simulink model "g1_walking"  (R2025b)
settings: Solver=daessc  StartTime=0.0  StopTime=4.8  MaxStep=0.0005  RelTol=1e-6  AbsTol=1e-8
model workspace (MAT data in the model file):
  g1_base_p0 = [0; 0; 0.8]
  g1_base_rpy0 = [0; 0; 0]
  g1_command_height = 0.8
  g1_forward_command = 0.1
  g1_gravity = [0 0 -9.81]
  g1_q0 = [-0.05 0 0 -0.05 0 0 0.1 0 0 0 0 0 ... (29 elements, 29x1)]
  g1_qd0 = [0 0 0 0 0 0 0 0 0 0 0 0 ... (29 elements, 29x1)]
  g1_standing = 0
values from neighbouring files (symbols this model uses):
  g1_action_Ts = 0.002    [g1_data.sldd]
  g1_contact_threshold = 1.0    [g1_data.sldd]
  g1_cop_threshold = 5.0    [g1_data.sldd]
  g1_drive_Ts = 0.0005    [g1_data.sldd]
  g1_ground_height = 0.0    [g1_data.sldd]
  g1_limits = -0.87267 -0.2618 -1.0472 -2.5307 -0.5236 -2.7576 -0.087267 -3.0892 -1.5882 -2.618 -1.614429558 -1.972222054 -1.614429558 -0.87267 -0.2618 -1.0472 -2.5307 -2.9671 -2.7576 -0.087267 -3.0892 -2.2515 -2.618 -1.614429558 -1.972222054 -1.614429558 -0.52 -0.52 -2.618 0.5236 0.2618 2.0944 2.8798 2.9671 2.7576 2.8798 2.6704 2.2515 2.618 1.614429558 1.972222054 1.614429558 0.5236 0.2618 2.0944 2.8798 0.5236    [g1_data.sldd]
  g1_tau_max = 50.0 50.0 25.0 88.0 88.0 88.0 139.0 25.0 25.0 25.0 5.0 25.0 5.0 50.0 50.0 25.0 88.0 88.0 88.0 139.0 25.0 25.0 25.0 5.0 25.0 5.0 50.0 50.0 88.0    [g1_data.sldd]
undefined symbols (not defined in the file or in its folder): X, Y, Z
libraries: sm_lib x336, nesl_utility x122, simulink x1
(part 2 of 7)

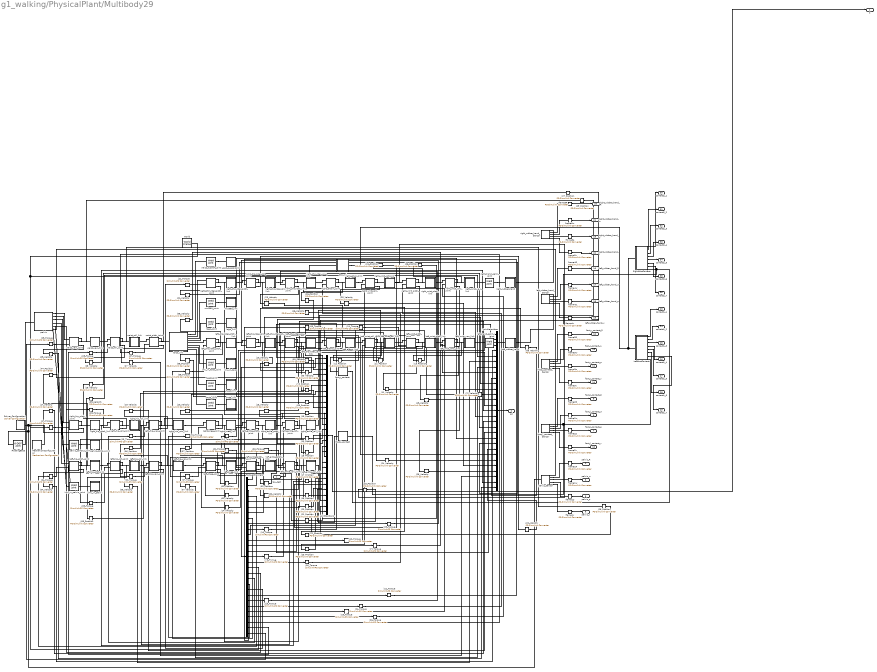
== system g1_walking/PhysicalPlant/Multibody29 ==
  tau_test : Inport  PortDimensions=29
  FloatingBase : sm_lib/Joints/6-DOF Joint  JointMode=Normal  CompositeWrenchDir=FollowerOnBase  CompositeWrenchFrame=BaseFrame  SenseConstraintForce=off  SenseConstraintTorque=off  SenseTotalForce=off  SenseTotalTorque=off  PxPositionTargetSpecify=on  PxPositionTargetPriority=High  PxPositionTargetValue=g1_base_p0(1)  PxPositionTargetValueUnits=m  PxVelocityTargetSpecify=on  PxVelocityTargetPriority=High  PxVelocityTargetValue=0  PxVelocityTargetValueUnits=m/s  PxEquilibriumPosition=0  PxEquilibriumPositionUnits=m  PxSpringStiffness=0  PxSpringStiffnessUnits=N/m  PxDampingCoefficient=0  PxDampingCoefficientUnits=N/(m/s)  PxLowerLimitSpecify=off  PxLowerLimitBound=-1  PxLowerLimitBoundUnits=m  PxLowerLimitStiffness=1e6  PxLowerLimitStiffnessUnits=N/m  PxLowerLimitDamping=1e3  PxLowerLimitDampingUnits=N/(m/s)  PxLowerLimitTransitionRegionWidth=1e-4  PxLowerLimitTransitionRegionWidthUnits=m  PxUpperLimitSpecify=off  PxUpperLimitBound=1  PxUpperLimitBoundUnits=m  PxUpperLimitStiffness=1e6  PxUpperLimitStiffnessUnits=N/m  PxUpperLimitDamping=1e3  PxUpperLimitDampingUnits=N/(m/s)  PxUpperLimitTransitionRegionWidth=1e-4  PxUpperLimitTransitionRegionWidthUnits=m  PxTorqueActuationMode=NoTorque  PxMotionActuationMode=ComputedMotion  PxSensePosition=off  PxSenseVelocity=off  PxSenseAcceleration=off  PxSenseTorqueForce=off  PxSenseLowerLimitTorqueForce=off  PxSenseUpperLimitTorqueForce=off  PyPositionTargetSpecify=on  PyPositionTargetPriority=High  PyPositionTargetValue=g1_base_p0(2)  PyPositionTargetValueUnits=m  PyVelocityTargetSpecify=on  PyVelocityTargetPriority=High  PyVelocityTargetValue=0  PyVelocityTargetValueUnits=m/s  PyEquilibriumPosition=0  PyEquilibriumPositionUnits=m  PySpringStiffness=0  PySpringStiffnessUnits=N/m  PyDampingCoefficient=0  PyDampingCoefficientUnits=N/(m/s)  PyLowerLimitSpecify=off  PyLowerLimitBound=-1  PyLowerLimitBoundUnits=m  PyLowerLimitStiffness=1e6  PyLowerLimitStiffnessUnits=N/m  PyLowerLimitDamping=1e3  PyLowerLimitDampingUnits=N/(m/s)  PyLowerLimitTransitionRegionWidth=1e-4  PyLowerLimitTransitionRegionWidthUnits=m  PyUpperLimitSpecify=off  PyUpperLimitBound=1  PyUpperLimitBoundUnits=m  PyUpperLimitStiffness=1e6  PyUpperLimitStiffnessUnits=N/m  PyUpperLimitDamping=1e3  PyUpperLimitDampingUnits=N/(m/s)  PyUpperLimitTransitionRegionWidth=1e-4  PyUpperLimitTransitionRegionWidthUnits=m  PyTorqueActuationMode=NoTorque  PyMotionActuationMode=ComputedMotion  PySensePosition=off  PySenseVelocity=off  PySenseAcceleration=off  PySenseTorqueForce=off  PySenseLowerLimitTorqueForce=off  PySenseUpperLimitTorqueForce=off  PzPositionTargetSpecify=on  PzPositionTargetPriority=High  PzPositionTargetValue=g1_base_p0(3)  PzPositionTargetValueUnits=m  PzVelocityTargetSpecify=on  PzVelocityTargetPriority=High  PzVelocityTargetValue=0  PzVelocityTargetValueUnits=m/s  PzEquilibriumPosition=0  PzEquilibriumPositionUnits=m  PzSpringStiffness=0  PzSpringStiffnessUnits=N/m  PzDampingCoefficient=0  PzDampingCoefficientUnits=N/(m/s)  PzLowerLimitSpecify=off  PzLowerLimitBound=-1  PzLowerLimitBoundUnits=m  PzLowerLimitStiffness=1e6  PzLowerLimitStiffnessUnits=N/m  PzLowerLimitDamping=1e3  PzLowerLimitDampingUnits=N/(m/s)  PzLowerLimitTransitionRegionWidth=1e-4  PzLowerLimitTransitionRegionWidthUnits=m  PzUpperLimitSpecify=off  PzUpperLimitBound=1  PzUpperLimitBoundUnits=m  PzUpperLimitStiffness=1e6  PzUpperLimitStiffnessUnits=N/m  PzUpperLimitDamping=1e3  PzUpperLimitDampingUnits=N/(m/s)  PzUpperLimitTransitionRegionWidth=1e-4  PzUpperLimitTransitionRegionWidthUnits=m  PzTorqueActuationMode=NoTorque  PzMotionActuationMode=ComputedMotion  PzSensePosition=off  PzSenseVelocity=off  PzSenseAcceleration=off  PzSenseTorqueForce=off  PzSenseLowerLimitTorqueForce=off  PzSenseUpperLimitTorqueForce=off  SphPositionTargetSpecify=on  SphPositionTargetPriority=High  SphPositionTargetRotationMethod=RotationSequence  SphPositionTargetFollAlignAxisA=+X  SphPositionTargetBaseAlignAxisA=+Y  SphPositionTargetFollAlignAxisB=+Y  SphPositionTargetBaseAlignAxisB=+Z  SphPositionTargetRotationStandardAxis=+Z  SphPositionTargetRotationAngle=0  SphPositionTargetRotationAngleUnits=deg  SphPositionTargetRotationArbitraryAxis=[0 0 1]  SphPositionTargetRotationSequenceAxes=FollowerAxes  SphPositionTargetRotationSequence=ZYX  SphPositionTargetRotationSequenceAngles=g1_base_rpy0([3 2 1])  SphPositionTargetRotationSequenceAnglesUnits=rad  SphPositionTargetRotationMatrix=[1 0 0;0 1 0;0 0 1]  SphPositionTargetQuaternion=[1 0 0 0]  SphVelocityTargetSpecify=on  SphVelocityTargetPriority=High  SphVelocityTargetValue=[0 0 0]  SphVelocityTargetValueUnits=rad/s  SphVelocityTargetInFollowerFrame=on  SphEqPosRotationMethod=None  SphEqPosFollAlignAxisA=+X  SphEqPosBaseAlignAxisA=+Y  SphEqPosFollAlignAxisB=+Y  SphEqPosBaseAlignAxisB=+Z  SphEqPosRotationStandardAxis=+Z  SphEqPosRotationAngle=0  SphEqPosRotationAngleUnits=deg  SphEqPosRotationArbitraryAxis=[0 0 1]  SphEqPosRotationSequenceAxes=FollowerAxes  SphEqPosRotationSequence=XYX  SphEqPosRotationSequenceAngles=[0 0 0]  SphEqPosRotationSequenceAnglesUnits=deg  SphEqPosRotationMatrix=[1 0 0;0 1 0;0 0 1]  SphEqPosQuaternion=[1 0 0 0]  SphSpringStiffness=0  SphSpringStiffnessUnits=N*m/deg  SphDampingCoefficient=0  SphDampingCoefficientUnits=N*m/(deg/s)  SphLowerLimitSpecify=off  SphLowerLimitBound=15  SphLowerLimitBoundUnits=deg  SphLowerLimitStiffness=1e4  SphLowerLimitStiffnessUnits=N*m/deg  SphLowerLimitDamping=10  SphLowerLimitDampingUnits=N*m/(deg/s)  SphLowerLimitTransitionRegionWidth=0.1  SphLowerLimitTransitionRegionWidthUnits=deg  SphUpperLimitSpecify=off  SphUpperLimitBound=45  SphUpperLimitBoundUnits=deg  SphUpperLimitStiffness=1e4  SphUpperLimitStiffnessUnits=N*m/deg  SphUpperLimitDamping=10  SphUpperLimitDampingUnits=N*m/(deg/s)  SphUpperLimitTransitionRegionWidth=0.1  SphUpperLimitTransitionRegionWidthUnits=deg  SphTorqueActuationMode=NoTorque  SphActuateTorqueX=off  SphActuateTorqueY=off  SphActuateTorqueZ=off  SphActuateTorque=off  SphActuationFrame=BaseFrame  SphSensePosition=off  SphSenseVelocityX=off  SphSenseVelocityY=off  SphSenseVelocityZ=off  SphSenseVelocity=off  SphSenseAccelerationX=off  SphSenseAccelerationY=off  SphSenseAccelerationZ=off  SphSenseAcceleration=off  SphSenseLowerLimitTorqueMag=off  SphSenseUpperLimitTorqueMag=off  SphSensingFrame=BaseFrame
  Ground : Subsystem
  JointPositions : Mux  Inputs=29
  JointVelocities : Mux  Inputs=29
  LeftFootContact : Subsystem
  MechanismConfiguration : sm_lib/Utilities/Mechanism Configuration  UniformGravity=Constant  GravityVector=g1_gravity  GravityVectorUnits=m/s^2  LinearizationDelta=0.001  JointModeTransitionNonlinearIterations=2
  RightFootContact : Subsystem
  Solver_Configuration : nesl_utility/Solver Configuration  PhysicalDomain=network_engine_domain  SubClassName=solver  LeftPortType=input  RightPortType=generic  Tones=[]  Harmonics=[]  SimulateNoise=off  Profile=off  UseLocalSampling=off  EnableSwitchedLinearOptims=on  FrequencyDomain=off  UseCCode=off  RelTol=0.001  AbsTol=0.001  MinStep=1e-09  ToWorkspace=off  RevertToSquareIcSolve=off  NumHomotopyIterations=100  PhasorMode=off  PhasorModeNumHarmonics=1  ConsistencySolver=NEWTON_XTOL_AFTER_FTOL  IndexReductionMethod=DerivativeReplacement  DoDC=off  ResidualTolerance=1e-09  ConsistencyTolSource=GLOBAL  ConsistencyAbsTol=0.001  ConsistencyRelTol=0.001  ConsistencyTolFactor=0.001  UseLocalSolver=off  LocalSolverChoice=NE_BACKWARD_EULER_ADVANCER  ResolveIndetEquations=on  FunctionEvalNumThread=1  LocalSolverSampleTime=0.001  DoFixedCost=off  MaxNonlinIter=3  MaxModeIter=2  ComputeImpulses=off  ImpulseIterations=2  LinearAlgebra=auto  LinearAlgebraNumThread=0  EquationFormulation=NE_TIME_EF  DelaysMemoryBudget=1024  AutomaticFiltering=on  FilteringTimeConstant=0.001  PartitionStorageMethod=AS_NEEDED  PartitionMemoryBudget=1024  PartitionMethod=ROBUST  MultibodyUseLocalSolver=off  MultibodyLocalSolverChoice=ODE1  MultibodyLocalSolverSampleTime=0.001
  TorqueChannels : Demux  Outputs=29
  World : sm_lib/Frames and Transforms/World Frame
  d435_joint : sm_lib/Joints/Weld Joint  JointMode=Normal  CompositeWrenchDir=FollowerOnBase  CompositeWrenchFrame=BaseFrame  SenseConstraintForce=off  SenseConstraintTorque=off  SenseTotalForce=off  SenseTotalTorque=off
  d435_link : Subsystem
  foot_l_contact : sm_lib/Frames and Transforms/Rigid Transform  RotationMethod=None  FollAlignAxisA=+X  BaseAlignAxisA=+Y  FollAlignAxisB=+Y  BaseAlignAxisB=+Z  RotationStandardAxis=+Z  RotationAngle=0  RotationAngleUnits=deg  RotationArbitraryAxis=[0 0 1]  RotationSequenceAxes=FollowerAxes  RotationSequence=XYX  RotationSequenceAngles=[0 0 0]  RotationSequenceAnglesUnits=deg  RotationMatrix=[1 0 0;0 1 0;0 0 1]  Quaternion=[1 0 0 0]  TranslationMethod=Cartesian  TranslationCartesianOffset=g1_foot_offset  TranslationCartesianOffsetUnits=m  TranslationStandardAxis=+Z  TranslationStandardOffset=0  TranslationStandardOffsetUnits=m  TranslationROffset=0  TranslationROffsetUnits=m  TranslationThetaOffset=0  TranslationThetaOffsetUnits=deg  TranslationZOffset=0  TranslationZOffsetUnits=m
  foot_l_contact_Sensor : sm_lib/Frames and Transforms/Transform Sensor  MeasurementFrame=World  RotationSequence=XYX  SenseAngle=off  SenseAxis=off  SenseQ=off  SenseR=on  SenseRotationSequence=off  SenseOmegaX=off  SenseOmegaY=off  SenseOmegaZ=off  SenseOmega=on  SenseQDot=off  SenseRDot=off  SenseRotationSequenceDot=off  SenseAlphaX=off  SenseAlphaY=off  SenseAlphaZ=off  SenseAlpha=off  SenseQDDot=off  SenseRDDot=off  SenseX=off  SenseY=off  SenseZ=off  SenseXYZ=on  SenseRad=off  SenseAzim=off  SenseDist=off  SenseInc=off  SenseXDot=off  SenseYDot=off  SenseZDot=off  SenseXYZDot=on  SenseRadDot=off  SenseAzimDot=off  SenseDistDot=off  SenseIncDot=off  SenseXDDot=off  SenseYDDot=off  SenseZDDot=off  SenseXYZDDot=off  SenseRadDDot=off  SenseAzimDDot=off  SenseDistDDot=off  SenseIncDDot=off
  foot_r_contact : sm_lib/Frames and Transforms/Rigid Transform  RotationMethod=None  FollAlignAxisA=+X  BaseAlignAxisA=+Y  FollAlignAxisB=+Y  BaseAlignAxisB=+Z  RotationStandardAxis=+Z  RotationAngle=0  RotationAngleUnits=deg  RotationArbitraryAxis=[0 0 1]  RotationSequenceAxes=FollowerAxes  RotationSequence=XYX  RotationSequenceAngles=[0 0 0]  RotationSequenceAnglesUnits=deg  RotationMatrix=[1 0 0;0 1 0;0 0 1]  Quaternion=[1 0 0 0]  TranslationMethod=Cartesian  TranslationCartesianOffset=g1_foot_offset  TranslationCartesianOffsetUnits=m  TranslationStandardAxis=+Z  TranslationStandardOffset=0  TranslationStandardOffsetUnits=m  TranslationROffset=0  TranslationROffsetUnits=m  TranslationThetaOffset=0  TranslationThetaOffsetUnits=deg  TranslationZOffset=0  TranslationZOffsetUnits=m
  foot_r_contact_Sensor : sm_lib/Frames and Transforms/Transform Sensor  MeasurementFrame=World  RotationSequence=XYX  SenseAngle=off  SenseAxis=off  SenseQ=off  SenseR=on  SenseRotationSequence=off  SenseOmegaX=off  SenseOmegaY=off  SenseOmegaZ=off  SenseOmega=on  SenseQDot=off  SenseRDot=off  SenseRotationSequenceDot=off  SenseAlphaX=off  SenseAlphaY=off  SenseAlphaZ=off  SenseAlpha=off  SenseQDDot=off  SenseRDDot=off  SenseX=off  SenseY=off  SenseZ=off  SenseXYZ=on  SenseRad=off  SenseAzim=off  SenseDist=off  SenseInc=off  SenseXDot=off  SenseYDot=off  SenseZDot=off  SenseXYZDot=on  SenseRadDot=off  SenseAzimDot=off  SenseDistDot=off  SenseIncDot=off  SenseXDDot=off  SenseYDDot=off  SenseZDDot=off  SenseXYZDDot=off  SenseRadDDot=off  SenseAzimDDot=off  SenseDistDDot=off  SenseIncDDot=off
  frame1R : nesl_utility/PS-Simulink Converter  PhysicalDomain=network_engine_domain  SubClassName=ps_output  LeftPortType=input  RightPortType=output  PseudoPeriodic=off  Frequencies=[]  VectorFormat=inherit  Unit=1  AffineConversion=off
  frame1p : nesl_utility/PS-Simulink Converter  PhysicalDomain=network_engine_domain  SubClassName=ps_output  LeftPortType=input  RightPortType=output  PseudoPeriodic=off  Frequencies=[]  VectorFormat=inherit  Unit=m  AffineConversion=off
  frame1v : nesl_utility/PS-Simulink Converter  PhysicalDomain=network_engine_domain  SubClassName=ps_output  LeftPortType=input  RightPortType=output  PseudoPeriodic=off  Frequencies=[]  VectorFormat=inherit  Unit=m/s  AffineConversion=off
  frame1w : nesl_utility/PS-Simulink Converter  PhysicalDomain=network_engine_domain  SubClassName=ps_output  LeftPortType=input  RightPortType=output  PseudoPeriodic=off  Frequencies=[]  VectorFormat=inherit  Unit=rad/s  AffineConversion=off
  frame2R : nesl_utility/PS-Simulink Converter  PhysicalDomain=network_engine_domain  SubClassName=ps_output  LeftPortType=input  RightPortType=output  PseudoPeriodic=off  Frequencies=[]  VectorFormat=inherit  Unit=1  AffineConversion=off
  frame2p : nesl_utility/PS-Simulink Converter  PhysicalDomain=network_engine_domain  SubClassName=ps_output  LeftPortType=input  RightPortType=output  PseudoPeriodic=off  Frequencies=[]  VectorFormat=inherit  Unit=m  AffineConversion=off
  frame2v : nesl_utility/PS-Simulink Converter  PhysicalDomain=network_engine_domain  SubClassName=ps_output  LeftPortType=input  RightPortType=output  PseudoPeriodic=off  Frequencies=[]  VectorFormat=inherit  Unit=m/s  AffineConversion=off
  frame2w : nesl_utility/PS-Simulink Converter  PhysicalDomain=network_engine_domain  SubClassName=ps_output  LeftPortType=input  RightPortType=output  PseudoPeriodic=off  Frequencies=[]  VectorFormat=inherit  Unit=rad/s  AffineConversion=off
  frame3R : nesl_utility/PS-Simulink Converter  PhysicalDomain=network_engine_domain  SubClassName=ps_output  LeftPortType=input  RightPortType=output  PseudoPeriodic=off  Frequencies=[]  VectorFormat=inherit  Unit=1  AffineConversion=off
  frame3p : nesl_utility/PS-Simulink Converter  PhysicalDomain=network_engine_domain  SubClassName=ps_output  LeftPortType=input  RightPortType=output  PseudoPeriodic=off  Frequencies=[]  VectorFormat=inherit  Unit=m  AffineConversion=off
  frame3v : nesl_utility/PS-Simulink Converter  PhysicalDomain=network_engine_domain  SubClassName=ps_output  LeftPortType=input  RightPortType=output  PseudoPeriodic=off  Frequencies=[]  VectorFormat=inherit  Unit=m/s  AffineConversion=off
  frame3w : nesl_utility/PS-Simulink Converter  PhysicalDomain=network_engine_domain  SubClassName=ps_output  LeftPortType=input  RightPortType=output  PseudoPeriodic=off  Frequencies=[]  VectorFormat=inherit  Unit=rad/s  AffineConversion=off
  frame4R : nesl_utility/PS-Simulink Converter  PhysicalDomain=network_engine_domain  SubClassName=ps_output  LeftPortType=input  RightPortType=output  PseudoPeriodic=off  Frequencies=[]  VectorFormat=inherit  Unit=1  AffineConversion=off
  frame4p : nesl_utility/PS-Simulink Converter  PhysicalDomain=network_engine_domain  SubClassName=ps_output  LeftPortType=input  RightPortType=output  PseudoPeriodic=off  Frequencies=[]  VectorFormat=inherit  Unit=m  AffineConversion=off
  frame4v : nesl_utility/PS-Simulink Converter  PhysicalDomain=network_engine_domain  SubClassName=ps_output  LeftPortType=input  RightPortType=output  PseudoPeriodic=off  Frequencies=[]  VectorFormat=inherit  Unit=m/s  AffineConversion=off
  frame4w : nesl_utility/PS-Simulink Converter  PhysicalDomain=network_engine_domain  SubClassName=ps_output  LeftPortType=input  RightPortType=output  PseudoPeriodic=off  Frequencies=[]  VectorFormat=inherit  Unit=rad/s  AffineConversion=off
  frame5R : nesl_utility/PS-Simulink Converter  PhysicalDomain=network_engine_domain  SubClassName=ps_output  LeftPortType=input  RightPortType=output  PseudoPeriodic=off  Frequencies=[]  VectorFormat=inherit  Unit=1  AffineConversion=off
  frame5p : nesl_utility/PS-Simulink Converter  PhysicalDomain=network_engine_domain  SubClassName=ps_output  LeftPortType=input  RightPortType=output  PseudoPeriodic=off  Frequencies=[]  VectorFormat=inherit  Unit=m  AffineConversion=off
  frame5v : nesl_utility/PS-Simulink Converter  PhysicalDomain=network_engine_domain  SubClassName=ps_output  LeftPortType=input  RightPortType=output  PseudoPeriodic=off  Frequencies=[]  VectorFormat=inherit  Unit=m/s  AffineConversion=off
  frame5w : nesl_utility/PS-Simulink Converter  PhysicalDomain=network_engine_domain  SubClassName=ps_output  LeftPortType=input  RightPortType=output  PseudoPeriodic=off  Frequencies=[]  VectorFormat=inherit  Unit=rad/s  AffineConversion=off
  head_joint : sm_lib/Joints/Weld Joint  JointMode=Normal  CompositeWrenchDir=FollowerOnBase  CompositeWrenchFrame=BaseFrame  SenseConstraintForce=off  SenseConstraintTorque=off  SenseTotalForce=off  SenseTotalTorque=off
  head_link : Subsystem
  imu_in_pelvis : Subsystem
  imu_in_pelvis_joint : sm_lib/Joints/Weld Joint  JointMode=Normal  CompositeWrenchDir=FollowerOnBase  CompositeWrenchFrame=BaseFrame  SenseConstraintForce=off  SenseConstraintTorque=off  SenseTotalForce=off  SenseTotalTorque=off
  imu_in_torso : Subsystem
  imu_in_torso_joint : sm_lib/Joints/Weld Joint  JointMode=Normal  CompositeWrenchDir=FollowerOnBase  CompositeWrenchFrame=BaseFrame  SenseConstraintForce=off  SenseConstraintTorque=off  SenseTotalForce=off  SenseTotalTorque=off
  j01_Position : nesl_utility/PS-Simulink Converter  PhysicalDomain=network_engine_domain  SubClassName=ps_output  LeftPortType=input  RightPortType=output  PseudoPeriodic=off  Frequencies=[]  VectorFormat=inherit  Unit=rad  AffineConversion=off
  j01_Torque : nesl_utility/Simulink-PS Converter  PhysicalDomain=network_engine_domain  SubClassName=ps_input  LeftPortType=input  RightPortType=output  PseudoPeriodic=off  Frequencies=[]  NoiseDistribution=none  NoiseParameters=[]  Unit=N*m  AffineConversion=off  FilteringAndDerivatives=provide  SimscapeFilterOrder=1  InputFilterTimeConstant=0.001  UdotUserProvided=0
  j01_Velocity : nesl_utility/PS-Simulink Converter  PhysicalDomain=network_engine_domain  SubClassName=ps_output  LeftPortType=input  RightPortType=output  PseudoPeriodic=off  Frequencies=[]  VectorFormat=inherit  Unit=rad/s  AffineConversion=off
  j02_Position : nesl_utility/PS-Simulink Converter  PhysicalDomain=network_engine_domain  SubClassName=ps_output  LeftPortType=input  RightPortType=output  PseudoPeriodic=off  Frequencies=[]  VectorFormat=inherit  Unit=rad  AffineConversion=off
  j02_Torque : nesl_utility/Simulink-PS Converter  PhysicalDomain=network_engine_domain  SubClassName=ps_input  LeftPortType=input  RightPortType=output  PseudoPeriodic=off  Frequencies=[]  NoiseDistribution=none  NoiseParameters=[]  Unit=N*m  AffineConversion=off  FilteringAndDerivatives=provide  SimscapeFilterOrder=1  InputFilterTimeConstant=0.001  UdotUserProvided=0
  j02_Velocity : nesl_utility/PS-Simulink Converter  PhysicalDomain=network_engine_domain  SubClassName=ps_output  LeftPortType=input  RightPortType=output  PseudoPeriodic=off  Frequencies=[]  VectorFormat=inherit  Unit=rad/s  AffineConversion=off
  j03_Position : nesl_utility/PS-Simulink Converter  PhysicalDomain=network_engine_domain  SubClassName=ps_output  LeftPortType=input  RightPortType=output  PseudoPeriodic=off  Frequencies=[]  VectorFormat=inherit  Unit=rad  AffineConversion=off
  j03_Torque : nesl_utility/Simulink-PS Converter  PhysicalDomain=network_engine_domain  SubClassName=ps_input  LeftPortType=input  RightPortType=output  PseudoPeriodic=off  Frequencies=[]  NoiseDistribution=none  NoiseParameters=[]  Unit=N*m  AffineConversion=off  FilteringAndDerivatives=provide  SimscapeFilterOrder=1  InputFilterTimeConstant=0.001  UdotUserProvided=0
  j03_Velocity : nesl_utility/PS-Simulink Converter  PhysicalDomain=network_engine_domain  SubClassName=ps_output  LeftPortType=input  RightPortType=output  PseudoPeriodic=off  Frequencies=[]  VectorFormat=inherit  Unit=rad/s  AffineConversion=off
  j04_Position : nesl_utility/PS-Simulink Converter  PhysicalDomain=network_engine_domain  SubClassName=ps_output  LeftPortType=input  RightPortType=output  PseudoPeriodic=off  Frequencies=[]  VectorFormat=inherit  Unit=rad  AffineConversion=off
  j04_Torque : nesl_utility/Simulink-PS Converter  PhysicalDomain=network_engine_domain  SubClassName=ps_input  LeftPortType=input  RightPortType=output  PseudoPeriodic=off  Frequencies=[]  NoiseDistribution=none  NoiseParameters=[]  Unit=N*m  AffineConversion=off  FilteringAndDerivatives=provide  SimscapeFilterOrder=1  InputFilterTimeConstant=0.001  UdotUserProvided=0
  j04_Velocity : nesl_utility/PS-Simulink Converter  PhysicalDomain=network_engine_domain  SubClassName=ps_output  LeftPortType=input  RightPortType=output  PseudoPeriodic=off  Frequencies=[]  VectorFormat=inherit  Unit=rad/s  AffineConversion=off
  j05_Position : nesl_utility/PS-Simulink Converter  PhysicalDomain=network_engine_domain  SubClassName=ps_output  LeftPortType=input  RightPortType=output  PseudoPeriodic=off  Frequencies=[]  VectorFormat=inherit  Unit=rad  AffineConversion=off
  j05_Torque : nesl_utility/Simulink-PS Converter  PhysicalDomain=network_engine_domain  SubClassName=ps_input  LeftPortType=input  RightPortType=output  PseudoPeriodic=off  Frequencies=[]  NoiseDistribution=none  NoiseParameters=[]  Unit=N*m  AffineConversion=off  FilteringAndDerivatives=provide  SimscapeFilterOrder=1  InputFilterTimeConstant=0.001  UdotUserProvided=0
  j05_Velocity : nesl_utility/PS-Simulink Converter  PhysicalDomain=network_engine_domain  SubClassName=ps_output  LeftPortType=input  RightPortType=output  PseudoPeriodic=off  Frequencies=[]  VectorFormat=inherit  Unit=rad/s  AffineConversion=off
  j06_Position : nesl_utility/PS-Simulink Converter  PhysicalDomain=network_engine_domain  SubClassName=ps_output  LeftPortType=input  RightPortType=output  PseudoPeriodic=off  Frequencies=[]  VectorFormat=inherit  Unit=rad  AffineConversion=off
  j06_Torque : nesl_utility/Simulink-PS Converter  PhysicalDomain=network_engine_domain  SubClassName=ps_input  LeftPortType=input  RightPortType=output  PseudoPeriodic=off  Frequencies=[]  NoiseDistribution=none  NoiseParameters=[]  Unit=N*m  AffineConversion=off  FilteringAndDerivatives=provide  SimscapeFilterOrder=1  InputFilterTimeConstant=0.001  UdotUserProvided=0
  j06_Velocity : nesl_utility/PS-Simulink Converter  PhysicalDomain=network_engine_domain  SubClassName=ps_output  LeftPortType=input  RightPortType=output  PseudoPeriodic=off  Frequencies=[]  VectorFormat=inherit  Unit=rad/s  AffineConversion=off
  j07_Position : nesl_utility/PS-Simulink Converter  PhysicalDomain=network_engine_domain  SubClassName=ps_output  LeftPortType=input  RightPortType=output  PseudoPeriodic=off  Frequencies=[]  VectorFormat=inherit  Unit=rad  AffineConversion=off
  j07_Torque : nesl_utility/Simulink-PS Converter  PhysicalDomain=network_engine_domain  SubClassName=ps_input  LeftPortType=input  RightPortType=output  PseudoPeriodic=off  Frequencies=[]  NoiseDistribution=none  NoiseParameters=[]  Unit=N*m  AffineConversion=off  FilteringAndDerivatives=provide  SimscapeFilterOrder=1  InputFilterTimeConstant=0.001  UdotUserProvided=0
  j07_Velocity : nesl_utility/PS-Simulink Converter  PhysicalDomain=network_engine_domain  SubClassName=ps_output  LeftPortType=input  RightPortType=output  PseudoPeriodic=off  Frequencies=[]  VectorFormat=inherit  Unit=rad/s  AffineConversion=off
  j08_Position : nesl_utility/PS-Simulink Converter  PhysicalDomain=network_engine_domain  SubClassName=ps_output  LeftPortType=input  RightPortType=output  PseudoPeriodic=off  Frequencies=[]  VectorFormat=inherit  Unit=rad  AffineConversion=off
  j08_Torque : nesl_utility/Simulink-PS Converter  PhysicalDomain=network_engine_domain  SubClassName=ps_input  LeftPortType=input  RightPortType=output  PseudoPeriodic=off  Frequencies=[]  NoiseDistribution=none  NoiseParameters=[]  Unit=N*m  AffineConversion=off  FilteringAndDerivatives=provide  SimscapeFilterOrder=1  InputFilterTimeConstant=0.001  UdotUserProvided=0
  j08_Velocity : nesl_utility/PS-Simulink Converter  PhysicalDomain=network_engine_domain  SubClassName=ps_output  LeftPortType=input  RightPortType=output  PseudoPeriodic=off  Frequencies=[]  VectorFormat=inherit  Unit=rad/s  AffineConversion=off
  j09_Position : nesl_utility/PS-Simulink Converter  PhysicalDomain=network_engine_domain  SubClassName=ps_output  LeftPortType=input  RightPortType=output  PseudoPeriodic=off  Frequencies=[]  VectorFormat=inherit  Unit=rad  AffineConversion=off
  j09_Torque : nesl_utility/Simulink-PS Converter  PhysicalDomain=network_engine_domain  SubClassName=ps_input  LeftPortType=input  RightPortType=output  PseudoPeriodic=off  Frequencies=[]  NoiseDistribution=none  NoiseParameters=[]  Unit=N*m  AffineConversion=off  FilteringAndDerivatives=provide  SimscapeFilterOrder=1  InputFilterTimeConstant=0.001  UdotUserProvided=0
  j09_Velocity : nesl_utility/PS-Simulink Converter  PhysicalDomain=network_engine_domain  SubClassName=ps_output  LeftPortType=input  RightPortType=output  PseudoPeriodic=off  Frequencies=[]  VectorFormat=inherit  Unit=rad/s  AffineConversion=off
  j10_Position : nesl_utility/PS-Simulink Converter  PhysicalDomain=network_engine_domain  SubClassName=ps_output  LeftPortType=input  RightPortType=output  PseudoPeriodic=off  Frequencies=[]  VectorFormat=inherit  Unit=rad  AffineConversion=off
  j10_Torque : nesl_utility/Simulink-PS Converter  PhysicalDomain=network_engine_domain  SubClassName=ps_input  LeftPortType=input  RightPortType=output  PseudoPeriodic=off  Frequencies=[]  NoiseDistribution=none  NoiseParameters=[]  Unit=N*m  AffineConversion=off  FilteringAndDerivatives=provide  SimscapeFilterOrder=1  InputFilterTimeConstant=0.001  UdotUserProvided=0
  j10_Velocity : nesl_utility/PS-Simulink Converter  PhysicalDomain=network_engine_domain  SubClassName=ps_output  LeftPortType=input  RightPortType=output  PseudoPeriodic=off  Frequencies=[]  VectorFormat=inherit  Unit=rad/s  AffineConversion=off
  j11_Position : nesl_utility/PS-Simulink Converter  PhysicalDomain=network_engine_domain  SubClassName=ps_output  LeftPortType=input  RightPortType=output  PseudoPeriodic=off  Frequencies=[]  VectorFormat=inherit  Unit=rad  AffineConversion=off
  j11_Torque : nesl_utility/Simulink-PS Converter  PhysicalDomain=network_engine_domain  SubClassName=ps_input  LeftPortType=input  RightPortType=output  PseudoPeriodic=off  Frequencies=[]  NoiseDistribution=none  NoiseParameters=[]  Unit=N*m  AffineConversion=off  FilteringAndDerivatives=provide  SimscapeFilterOrder=1  InputFilterTimeConstant=0.001  UdotUserProvided=0
  j11_Velocity : nesl_utility/PS-Simulink Converter  PhysicalDomain=network_engine_domain  SubClassName=ps_output  LeftPortType=input  RightPortType=output  PseudoPeriodic=off  Frequencies=[]  VectorFormat=inherit  Unit=rad/s  AffineConversion=off
  j12_Position : nesl_utility/PS-Simulink Converter  PhysicalDomain=network_engine_domain  SubClassName=ps_output  LeftPortType=input  RightPortType=output  PseudoPeriodic=off  Frequencies=[]  VectorFormat=inherit  Unit=rad  AffineConversion=off
  j12_Torque : nesl_utility/Simulink-PS Converter  PhysicalDomain=network_engine_domain  SubClassName=ps_input  LeftPortType=input  RightPortType=output  PseudoPeriodic=off  Frequencies=[]  NoiseDistribution=none  NoiseParameters=[]  Unit=N*m  AffineConversion=off  FilteringAndDerivatives=provide  SimscapeFilterOrder=1  InputFilterTimeConstant=0.001  UdotUserProvided=0
  j12_Velocity : nesl_utility/PS-Simulink Converter  PhysicalDomain=network_engine_domain  SubClassName=ps_output  LeftPortType=input  RightPortType=output  PseudoPeriodic=off  Frequencies=[]  VectorFormat=inherit  Unit=rad/s  AffineConversion=off
  j13_Position : nesl_utility/PS-Simulink Converter  PhysicalDomain=network_engine_domain  SubClassName=ps_output  LeftPortType=input  RightPortType=output  PseudoPeriodic=off  Frequencies=[]  VectorFormat=inherit  Unit=rad  AffineConversion=off
  j13_Torque : nesl_utility/Simulink-PS Converter  PhysicalDomain=network_engine_domain  SubClassName=ps_input  LeftPortType=input  RightPortType=output  PseudoPeriodic=off  Frequencies=[]  NoiseDistribution=none  NoiseParameters=[]  Unit=N*m  AffineConversion=off  FilteringAndDerivatives=provide  SimscapeFilterOrder=1  InputFilterTimeConstant=0.001  UdotUserProvided=0
  j13_Velocity : nesl_utility/PS-Simulink Converter  PhysicalDomain=network_engine_domain  SubClassName=ps_output  LeftPortType=input  RightPortType=output  PseudoPeriodic=off  Frequencies=[]  VectorFormat=inherit  Unit=rad/s  AffineConversion=off
  j14_Position : nesl_utility/PS-Simulink Converter  PhysicalDomain=network_engine_domain  SubClassName=ps_output  LeftPortType=input  RightPortType=output  PseudoPeriodic=off  Frequencies=[]  VectorFormat=inherit  Unit=rad  AffineConversion=off
  j14_Torque : nesl_utility/Simulink-PS Converter  PhysicalDomain=network_engine_domain  SubClassName=ps_input  LeftPortType=input  RightPortType=output  PseudoPeriodic=off  Frequencies=[]  NoiseDistribution=none  NoiseParameters=[]  Unit=N*m  AffineConversion=off  FilteringAndDerivatives=provide  SimscapeFilterOrder=1  InputFilterTimeConstant=0.001  UdotUserProvided=0
  j14_Velocity : nesl_utility/PS-Simulink Converter  PhysicalDomain=network_engine_domain  SubClassName=ps_output  LeftPortType=input  RightPortType=output  PseudoPeriodic=off  Frequencies=[]  VectorFormat=inherit  Unit=rad/s  AffineConversion=off
  j15_Position : nesl_utility/PS-Simulink Converter  PhysicalDomain=network_engine_domain  SubClassName=ps_output  LeftPortType=input  RightPortType=output  PseudoPeriodic=off  Frequencies=[]  VectorFormat=inherit  Unit=rad  AffineConversion=off
  j15_Torque : nesl_utility/Simulink-PS Converter  PhysicalDomain=network_engine_domain  SubClassName=ps_input  LeftPortType=input  RightPortType=output  PseudoPeriodic=off  Frequencies=[]  NoiseDistribution=none  NoiseParameters=[]  Unit=N*m  AffineConversion=off  FilteringAndDerivatives=provide  SimscapeFilterOrder=1  InputFilterTimeConstant=0.001  UdotUserProvided=0
  j15_Velocity : nesl_utility/PS-Simulink Converter  PhysicalDomain=network_engine_domain  SubClassName=ps_output  LeftPortType=input  RightPortType=output  PseudoPeriodic=off  Frequencies=[]  VectorFormat=inherit  Unit=rad/s  AffineConversion=off
  j16_Position : nesl_utility/PS-Simulink Converter  PhysicalDomain=network_engine_domain  SubClassName=ps_output  LeftPortType=input  RightPortType=output  PseudoPeriodic=off  Frequencies=[]  VectorFormat=inherit  Unit=rad  AffineConversion=off
  j16_Torque : nesl_utility/Simulink-PS Converter  PhysicalDomain=network_engine_domain  SubClassName=ps_input  LeftPortType=input  RightPortType=output  PseudoPeriodic=off  Frequencies=[]  NoiseDistribution=none  NoiseParameters=[]  Unit=N*m  AffineConversion=off  FilteringAndDerivatives=provide  SimscapeFilterOrder=1  InputFilterTimeConstant=0.001  UdotUserProvided=0
  j16_Velocity : nesl_utility/PS-Simulink Converter  PhysicalDomain=network_engine_domain  SubClassName=ps_output  LeftPortType=input  RightPortType=output  PseudoPeriodic=off  Frequencies=[]  VectorFormat=inherit  Unit=rad/s  AffineConversion=off
  j17_Position : nesl_utility/PS-Simulink Converter  PhysicalDomain=network_engine_domain  SubClassName=ps_output  LeftPortType=input  RightPortType=output  PseudoPeriodic=off  Frequencies=[]  VectorFormat=inherit  Unit=rad  AffineConversion=off
  j17_Torque : nesl_utility/Simulink-PS Converter  PhysicalDomain=network_engine_domain  SubClassName=ps_input  LeftPortType=input  RightPortType=output  PseudoPeriodic=off  Frequencies=[]  NoiseDistribution=none  NoiseParameters=[]  Unit=N*m  AffineConversion=off  FilteringAndDerivatives=provide  SimscapeFilterOrder=1  InputFilterTimeConstant=0.001  UdotUserProvided=0
  j17_Velocity : nesl_utility/PS-Simulink Converter  PhysicalDomain=network_engine_domain  SubClassName=ps_output  LeftPortType=input  RightPortType=output  PseudoPeriodic=off  Frequencies=[]  VectorFormat=inherit  Unit=rad/s  AffineConversion=off
  j18_Position : nesl_utility/PS-Simulink Converter  PhysicalDomain=network_engine_domain  SubClassName=ps_output  LeftPortType=input  RightPortType=output  PseudoPeriodic=off  Frequencies=[]  VectorFormat=inherit  Unit=rad  AffineConversion=off
  j18_Torque : nesl_utility/Simulink-PS Converter  PhysicalDomain=network_engine_domain  SubClassName=ps_input  LeftPortType=input  RightPortType=output  PseudoPeriodic=off  Frequencies=[]  NoiseDistribution=none  NoiseParameters=[]  Unit=N*m  AffineConversion=off  FilteringAndDerivatives=provide  SimscapeFilterOrder=1  InputFilterTimeConstant=0.001  UdotUserProvided=0
  j18_Velocity : nesl_utility/PS-Simulink Converter  PhysicalDomain=network_engine_domain  SubClassName=ps_output  LeftPortType=input  RightPortType=output  PseudoPeriodic=off  Frequencies=[]  VectorFormat=inherit  Unit=rad/s  AffineConversion=off
  j19_Position : nesl_utility/PS-Simulink Converter  PhysicalDomain=network_engine_domain  SubClassName=ps_output  LeftPortType=input  RightPortType=output  PseudoPeriodic=off  Frequencies=[]  VectorFormat=inherit  Unit=rad  AffineConversion=off
  j19_Torque : nesl_utility/Simulink-PS Converter  PhysicalDomain=network_engine_domain  SubClassName=ps_input  LeftPortType=input  RightPortType=output  PseudoPeriodic=off  Frequencies=[]  NoiseDistribution=none  NoiseParameters=[]  Unit=N*m  AffineConversion=off  FilteringAndDerivatives=provide  SimscapeFilterOrder=1  InputFilterTimeConstant=0.001  UdotUserProvided=0
  j19_Velocity : nesl_utility/PS-Simulink Converter  PhysicalDomain=network_engine_domain  SubClassName=ps_output  LeftPortType=input  RightPortType=output  PseudoPeriodic=off  Frequencies=[]  VectorFormat=inherit  Unit=rad/s  AffineConversion=off
  j20_Position : nesl_utility/PS-Simulink Converter  PhysicalDomain=network_engine_domain  SubClassName=ps_output  LeftPortType=input  RightPortType=output  PseudoPeriodic=off  Frequencies=[]  VectorFormat=inherit  Unit=rad  AffineConversion=off
  j20_Torque : nesl_utility/Simulink-PS Converter  PhysicalDomain=network_engine_domain  SubClassName=ps_input  LeftPortType=input  RightPortType=output  PseudoPeriodic=off  Frequencies=[]  NoiseDistribution=none  NoiseParameters=[]  Unit=N*m  AffineConversion=off  FilteringAndDerivatives=provide  SimscapeFilterOrder=1  InputFilterTimeConstant=0.001  UdotUserProvided=0
  j20_Velocity : nesl_utility/PS-Simulink Converter  PhysicalDomain=network_engine_domain  SubClassName=ps_output  LeftPortType=input  RightPortType=output  PseudoPeriodic=off  Frequencies=[]  VectorFormat=inherit  Unit=rad/s  AffineConversion=off
  j21_Position : nesl_utility/PS-Simulink Converter  PhysicalDomain=network_engine_domain  SubClassName=ps_output  LeftPortType=input  RightPortType=output  PseudoPeriodic=off  Frequencies=[]  VectorFormat=inherit  Unit=rad  AffineConversion=off
  j21_Torque : nesl_utility/Simulink-PS Converter  PhysicalDomain=network_engine_domain  SubClassName=ps_input  LeftPortType=input  RightPortType=output  PseudoPeriodic=off  Frequencies=[]  NoiseDistribution=none  NoiseParameters=[]  Unit=N*m  AffineConversion=off  FilteringAndDerivatives=provide  SimscapeFilterOrder=1  InputFilterTimeConstant=0.001  UdotUserProvided=0
  j21_Velocity : nesl_utility/PS-Simulink Converter  PhysicalDomain=network_engine_domain  SubClassName=ps_output  LeftPortType=input  RightPortType=output  PseudoPeriodic=off  Frequencies=[]  VectorFormat=inherit  Unit=rad/s  AffineConversion=off
  j22_Position : nesl_utility/PS-Simulink Converter  PhysicalDomain=network_engine_domain  SubClassName=ps_output  LeftPortType=input  RightPortType=output  PseudoPeriodic=off  Frequencies=[]  VectorFormat=inherit  Unit=rad  AffineConversion=off
  j22_Torque : nesl_utility/Simulink-PS Converter  PhysicalDomain=network_engine_domain  SubClassName=ps_input  LeftPortType=input  RightPortType=output  PseudoPeriodic=off  Frequencies=[]  NoiseDistribution=none  NoiseParameters=[]  Unit=N*m  AffineConversion=off  FilteringAndDerivatives=provide  SimscapeFilterOrder=1  InputFilterTimeConstant=0.001  UdotUserProvided=0
  j22_Velocity : nesl_utility/PS-Simulink Converter  PhysicalDomain=network_engine_domain  SubClassName=ps_output  LeftPortType=input  RightPortType=output  PseudoPeriodic=off  Frequencies=[]  VectorFormat=inherit  Unit=rad/s  AffineConversion=off
  j23_Position : nesl_utility/PS-Simulink Converter  PhysicalDomain=network_engine_domain  SubClassName=ps_output  LeftPortType=input  RightPortType=output  PseudoPeriodic=off  Frequencies=[]  VectorFormat=inherit  Unit=rad  AffineConversion=off
  j23_Torque : nesl_utility/Simulink-PS Converter  PhysicalDomain=network_engine_domain  SubClassName=ps_input  LeftPortType=input  RightPortType=output  PseudoPeriodic=off  Frequencies=[]  NoiseDistribution=none  NoiseParameters=[]  Unit=N*m  AffineConversion=off  FilteringAndDerivatives=provide  SimscapeFilterOrder=1  InputFilterTimeConstant=0.001  UdotUserProvided=0
  j23_Velocity : nesl_utility/PS-Simulink Converter  PhysicalDomain=network_engine_domain  SubClassName=ps_output  LeftPortType=input  RightPortType=output  PseudoPeriodic=off  Frequencies=[]  VectorFormat=inherit  Unit=rad/s  AffineConversion=off
  j24_Position : nesl_utility/PS-Simulink Converter  PhysicalDomain=network_engine_domain  SubClassName=ps_output  LeftPortType=input  RightPortType=output  PseudoPeriodic=off  Frequencies=[]  VectorFormat=inherit  Unit=rad  AffineConversion=off
  j24_Torque : nesl_utility/Simulink-PS Converter  PhysicalDomain=network_engine_domain  SubClassName=ps_input  LeftPortType=input  RightPortType=output  PseudoPeriodic=off  Frequencies=[]  NoiseDistribution=none  NoiseParameters=[]  Unit=N*m  AffineConversion=off  FilteringAndDerivatives=provide  SimscapeFilterOrder=1  InputFilterTimeConstant=0.001  UdotUserProvided=0
  j24_Velocity : nesl_utility/PS-Simulink Converter  PhysicalDomain=network_engine_domain  SubClassName=ps_output  LeftPortType=input  RightPortType=output  PseudoPeriodic=off  Frequencies=[]  VectorFormat=inherit  Unit=rad/s  AffineConversion=off
  j25_Position : nesl_utility/PS-Simulink Converter  PhysicalDomain=network_engine_domain  SubClassName=ps_output  LeftPortType=input  RightPortType=output  PseudoPeriodic=off  Frequencies=[]  VectorFormat=inherit  Unit=rad  AffineConversion=off
  j25_Torque : nesl_utility/Simulink-PS Converter  PhysicalDomain=network_engine_domain  SubClassName=ps_input  LeftPortType=input  RightPortType=output  PseudoPeriodic=off  Frequencies=[]  NoiseDistribution=none  NoiseParameters=[]  Unit=N*m  AffineConversion=off  FilteringAndDerivatives=provide  SimscapeFilterOrder=1  InputFilterTimeConstant=0.001  UdotUserProvided=0
  j25_Velocity : nesl_utility/PS-Simulink Converter  PhysicalDomain=network_engine_domain  SubClassName=ps_output  LeftPortType=input  RightPortType=output  PseudoPeriodic=off  Frequencies=[]  VectorFormat=inherit  Unit=rad/s  AffineConversion=off
  j26_Position : nesl_utility/PS-Simulink Converter  PhysicalDomain=network_engine_domain  SubClassName=ps_output  LeftPortType=input  RightPortType=output  PseudoPeriodic=off  Frequencies=[]  VectorFormat=inherit  Unit=rad  AffineConversion=off
  j26_Torque : nesl_utility/Simulink-PS Converter  PhysicalDomain=network_engine_domain  SubClassName=ps_input  LeftPortType=input  RightPortType=output  PseudoPeriodic=off  Frequencies=[]  NoiseDistribution=none  NoiseParameters=[]  Unit=N*m  AffineConversion=off  FilteringAndDerivatives=provide  SimscapeFilterOrder=1  InputFilterTimeConstant=0.001  UdotUserProvided=0
  j26_Velocity : nesl_utility/PS-Simulink Converter  PhysicalDomain=network_engine_domain  SubClassName=ps_output  LeftPortType=input  RightPortType=output  PseudoPeriodic=off  Frequencies=[]  VectorFormat=inherit  Unit=rad/s  AffineConversion=off
  j27_Position : nesl_utility/PS-Simulink Converter  PhysicalDomain=network_engine_domain  SubClassName=ps_output  LeftPortType=input  RightPortType=output  PseudoPeriodic=off  Frequencies=[]  VectorFormat=inherit  Unit=rad  AffineConversion=off
  j27_Torque : nesl_utility/Simulink-PS Converter  PhysicalDomain=network_engine_domain  SubClassName=ps_input  LeftPortType=input  RightPortType=output  PseudoPeriodic=off  Frequencies=[]  NoiseDistribution=none  NoiseParameters=[]  Unit=N*m  AffineConversion=off  FilteringAndDerivatives=provide  SimscapeFilterOrder=1  InputFilterTimeConstant=0.001  UdotUserProvided=0
  j27_Velocity : nesl_utility/PS-Simulink Converter  PhysicalDomain=network_engine_domain  SubClassName=ps_output  LeftPortType=input  RightPortType=output  PseudoPeriodic=off  Frequencies=[]  VectorFormat=inherit  Unit=rad/s  AffineConversion=off
  j28_Position : nesl_utility/PS-Simulink Converter  PhysicalDomain=network_engine_domain  SubClassName=ps_output  LeftPortType=input  RightPortType=output  PseudoPeriodic=off  Frequencies=[]  VectorFormat=inherit  Unit=rad  AffineConversion=off
  j28_Torque : nesl_utility/Simulink-PS Converter  PhysicalDomain=network_engine_domain  SubClassName=ps_input  LeftPortType=input  RightPortType=output  PseudoPeriodic=off  Frequencies=[]  NoiseDistribution=none  NoiseParameters=[]  Unit=N*m  AffineConversion=off  FilteringAndDerivatives=provide  SimscapeFilterOrder=1  InputFilterTimeConstant=0.001  UdotUserProvided=0
  j28_Velocity : nesl_utility/PS-Simulink Converter  PhysicalDomain=network_engine_domain  SubClassName=ps_output  LeftPortType=input  RightPortType=output  PseudoPeriodic=off  Frequencies=[]  VectorFormat=inherit  Unit=rad/s  AffineConversion=off
  j29_Position : nesl_utility/PS-Simulink Converter  PhysicalDomain=network_engine_domain  SubClassName=ps_output  LeftPortType=input  RightPortType=output  PseudoPeriodic=off  Frequencies=[]  VectorFormat=inherit  Unit=rad  AffineConversion=off
  j29_Torque : nesl_utility/Simulink-PS Converter  PhysicalDomain=network_engine_domain  SubClassName=ps_input  LeftPortType=input  RightPortType=output  PseudoPeriodic=off  Frequencies=[]  NoiseDistribution=none  NoiseParameters=[]  Unit=N*m  AffineConversion=off  FilteringAndDerivatives=provide  SimscapeFilterOrder=1  InputFilterTimeConstant=0.001  UdotUserProvided=0
  j29_Velocity : nesl_utility/PS-Simulink Converter  PhysicalDomain=network_engine_domain  SubClassName=ps_output  LeftPortType=input  RightPortType=output  PseudoPeriodic=off  Frequencies=[]  VectorFormat=inherit  Unit=rad/s  AffineConversion=off
  left_ankle_pitch_joint : sm_lib/Joints/Revolute Joint  JointMode=Normal  CompositeWrenchDir=FollowerOnBase  CompositeWrenchFrame=BaseFrame  SenseConstraintForce=off  SenseConstraintTorque=off  SenseTotalForce=off  SenseTotalTorque=off  PositionTargetSpecify=on  PositionTargetPriority=High  PositionTargetValue=g1_q0(1)  PositionTargetValueUnits=rad  VelocityTargetSpecify=on  VelocityTargetPriority=High  VelocityTargetValue=g1_qd0(1)  VelocityTargetValueUnits=rad/s  EquilibriumPosition=0  EquilibriumPositionUnits=deg  SpringStiffness=0  SpringStiffnessUnits=N*m/rad  DampingCoefficient=g1_damping  DampingCoefficientUnits=N*m/(rad/s)  LowerLimitSpecify=on  LowerLimitBound=g1_limits(1,1)  LowerLimitBoundUnits=rad  LowerLimitStiffness=g1_stop_k  LowerLimitStiffnessUnits=N*m/rad  LowerLimitDamping=g1_stop_d  LowerLimitDampingUnits=N*m/(rad/s)  LowerLimitTransitionRegionWidth=g1_stop_width  LowerLimitTransitionRegionWidthUnits=rad  UpperLimitSpecify=on  UpperLimitBound=g1_limits(1,2)  UpperLimitBoundUnits=rad  UpperLimitStiffness=g1_stop_k  UpperLimitStiffnessUnits=N*m/rad  UpperLimitDamping=g1_stop_d  UpperLimitDampingUnits=N*m/(rad/s)  UpperLimitTransitionRegionWidth=g1_stop_width  UpperLimitTransitionRegionWidthUnits=rad  TorqueActuationMode=InputTorque  MotionActuationMode=ComputedMotion  SensePosition=on  SenseVelocity=on  SenseAcceleration=off  SenseTorqueForce=off  SenseLowerLimitTorqueForce=off  SenseUpperLimitTorqueForce=off
  left_ankle_pitch_link : Subsystem
  left_ankle_roll_joint : sm_lib/Joints/Revolute Joint  JointMode=Normal  CompositeWrenchDir=FollowerOnBase  CompositeWrenchFrame=BaseFrame  SenseConstraintForce=off  SenseConstraintTorque=off  SenseTotalForce=off  SenseTotalTorque=off  PositionTargetSpecify=on  PositionTargetPriority=High  PositionTargetValue=g1_q0(2)  PositionTargetValueUnits=rad  VelocityTargetSpecify=on  VelocityTargetPriority=High  VelocityTargetValue=g1_qd0(2)  VelocityTargetValueUnits=rad/s  EquilibriumPosition=0  EquilibriumPositionUnits=deg  SpringStiffness=0  SpringStiffnessUnits=N*m/rad  DampingCoefficient=g1_damping  DampingCoefficientUnits=N*m/(rad/s)  LowerLimitSpecify=on  LowerLimitBound=g1_limits(2,1)  LowerLimitBoundUnits=rad  LowerLimitStiffness=g1_stop_k  LowerLimitStiffnessUnits=N*m/rad  LowerLimitDamping=g1_stop_d  LowerLimitDampingUnits=N*m/(rad/s)  LowerLimitTransitionRegionWidth=g1_stop_width  LowerLimitTransitionRegionWidthUnits=rad  UpperLimitSpecify=on  UpperLimitBound=g1_limits(2,2)  UpperLimitBoundUnits=rad  UpperLimitStiffness=g1_stop_k  UpperLimitStiffnessUnits=N*m/rad  UpperLimitDamping=g1_stop_d  UpperLimitDampingUnits=N*m/(rad/s)  UpperLimitTransitionRegionWidth=g1_stop_width  UpperLimitTransitionRegionWidthUnits=rad  TorqueActuationMode=InputTorque  MotionActuationMode=ComputedMotion  SensePosition=on  SenseVelocity=on  SenseAcceleration=off  SenseTorqueForce=off  SenseLowerLimitTorqueForce=off  SenseUpperLimitTorqueForce=off
  left_ankle_roll_link : Subsystem
  left_elbow_joint : sm_lib/Joints/Revolute Joint  JointMode=Normal  CompositeWrenchDir=FollowerOnBase  CompositeWrenchFrame=BaseFrame  SenseConstraintForce=off  SenseConstraintTorque=off  SenseTotalForce=off  SenseTotalTorque=off  PositionTargetSpecify=on  PositionTargetPriority=High  PositionTargetValue=g1_q0(3)  PositionTargetValueUnits=rad  VelocityTargetSpecify=on  VelocityTargetPriority=High  VelocityTargetValue=g1_qd0(3)  VelocityTargetValueUnits=rad/s  EquilibriumPosition=0  EquilibriumPositionUnits=deg  SpringStiffness=0  SpringStiffnessUnits=N*m/rad  DampingCoefficient=g1_damping  DampingCoefficientUnits=N*m/(rad/s)  LowerLimitSpecify=on  LowerLimitBound=g1_limits(3,1)  LowerLimitBoundUnits=rad  LowerLimitStiffness=g1_stop_k  LowerLimitStiffnessUnits=N*m/rad  LowerLimitDamping=g1_stop_d  LowerLimitDampingUnits=N*m/(rad/s)  LowerLimitTransitionRegionWidth=g1_stop_width  LowerLimitTransitionRegionWidthUnits=rad  UpperLimitSpecify=on  UpperLimitBound=g1_limits(3,2)  UpperLimitBoundUnits=rad  UpperLimitStiffness=g1_stop_k  UpperLimitStiffnessUnits=N*m/rad  UpperLimitDamping=g1_stop_d  UpperLimitDampingUnits=N*m/(rad/s)  UpperLimitTransitionRegionWidth=g1_stop_width  UpperLimitTransitionRegionWidthUnits=rad  TorqueActuationMode=InputTorque  MotionActuationMode=ComputedMotion  SensePosition=on  SenseVelocity=on  SenseAcceleration=off  SenseTorqueForce=off  SenseLowerLimitTorqueForce=off  SenseUpperLimitTorqueForce=off
  left_elbow_link : Subsystem
  left_hand_palm_joint : sm_lib/Joints/Weld Joint  JointMode=Normal  CompositeWrenchDir=FollowerOnBase  CompositeWrenchFrame=BaseFrame  SenseConstraintForce=off  SenseConstraintTorque=off  SenseTotalForce=off  SenseTotalTorque=off
  left_hip_pitch_joint : sm_lib/Joints/Revolute Joint  JointMode=Normal  CompositeWrenchDir=FollowerOnBase  CompositeWrenchFrame=BaseFrame  SenseConstraintForce=off  SenseConstraintTorque=off  SenseTotalForce=off  SenseTotalTorque=off  PositionTargetSpecify=on  PositionTargetPriority=High  PositionTargetValue=g1_q0(4)  PositionTargetValueUnits=rad  VelocityTargetSpecify=on  VelocityTargetPriority=High  VelocityTargetValue=g1_qd0(4)  VelocityTargetValueUnits=rad/s  EquilibriumPosition=0  EquilibriumPositionUnits=deg  SpringStiffness=0  SpringStiffnessUnits=N*m/rad  DampingCoefficient=g1_damping  DampingCoefficientUnits=N*m/(rad/s)  LowerLimitSpecify=on  LowerLimitBound=g1_limits(4,1)  LowerLimitBoundUnits=rad  LowerLimitStiffness=g1_stop_k  LowerLimitStiffnessUnits=N*m/rad  LowerLimitDamping=g1_stop_d  LowerLimitDampingUnits=N*m/(rad/s)  LowerLimitTransitionRegionWidth=g1_stop_width  LowerLimitTransitionRegionWidthUnits=rad  UpperLimitSpecify=on  UpperLimitBound=g1_limits(4,2)  UpperLimitBoundUnits=rad  UpperLimitStiffness=g1_stop_k  UpperLimitStiffnessUnits=N*m/rad  UpperLimitDamping=g1_stop_d  UpperLimitDampingUnits=N*m/(rad/s)  UpperLimitTransitionRegionWidth=g1_stop_width  UpperLimitTransitionRegionWidthUnits=rad  TorqueActuationMode=InputTorque  MotionActuationMode=ComputedMotion  SensePosition=on  SenseVelocity=on  SenseAcceleration=off  SenseTorqueForce=off  SenseLowerLimitTorqueForce=off  SenseUpperLimitTorqueForce=off
  left_hip_pitch_link : Subsystem
  left_hip_roll_joint : sm_lib/Joints/Revolute Joint  JointMode=Normal  CompositeWrenchDir=FollowerOnBase  CompositeWrenchFrame=BaseFrame  SenseConstraintForce=off  SenseConstraintTorque=off  SenseTotalForce=off  SenseTotalTorque=off  PositionTargetSpecify=on  PositionTargetPriority=High  PositionTargetValue=g1_q0(5)  PositionTargetValueUnits=rad  VelocityTargetSpecify=on  VelocityTargetPriority=High  VelocityTargetValue=g1_qd0(5)  VelocityTargetValueUnits=rad/s  EquilibriumPosition=0  EquilibriumPositionUnits=deg  SpringStiffness=0  SpringStiffnessUnits=N*m/rad  DampingCoefficient=g1_damping  DampingCoefficientUnits=N*m/(rad/s)  LowerLimitSpecify=on  LowerLimitBound=g1_limits(5,1)  LowerLimitBoundUnits=rad  LowerLimitStiffness=g1_stop_k  LowerLimitStiffnessUnits=N*m/rad  LowerLimitDamping=g1_stop_d  LowerLimitDampingUnits=N*m/(rad/s)  LowerLimitTransitionRegionWidth=g1_stop_width  LowerLimitTransitionRegionWidthUnits=rad  UpperLimitSpecify=on  UpperLimitBound=g1_limits(5,2)  UpperLimitBoundUnits=rad  UpperLimitStiffness=g1_stop_k  UpperLimitStiffnessUnits=N*m/rad  UpperLimitDamping=g1_stop_d  UpperLimitDampingUnits=N*m/(rad/s)  UpperLimitTransitionRegionWidth=g1_stop_width  UpperLimitTransitionRegionWidthUnits=rad  TorqueActuationMode=InputTorque  MotionActuationMode=ComputedMotion  SensePosition=on  SenseVelocity=on  SenseAcceleration=off  SenseTorqueForce=off  SenseLowerLimitTorqueForce=off  SenseUpperLimitTorqueForce=off
  left_hip_roll_link : Subsystem
  left_hip_yaw_joint : sm_lib/Joints/Revolute Joint  JointMode=Normal  CompositeWrenchDir=FollowerOnBase  CompositeWrenchFrame=BaseFrame  SenseConstraintForce=off  SenseConstraintTorque=off  SenseTotalForce=off  SenseTotalTorque=off  PositionTargetSpecify=on  PositionTargetPriority=High  PositionTargetValue=g1_q0(6)  PositionTargetValueUnits=rad  VelocityTargetSpecify=on  VelocityTargetPriority=High  VelocityTargetValue=g1_qd0(6)  VelocityTargetValueUnits=rad/s  EquilibriumPosition=0  EquilibriumPositionUnits=deg  SpringStiffness=0  SpringStiffnessUnits=N*m/rad  DampingCoefficient=g1_damping  DampingCoefficientUnits=N*m/(rad/s)  LowerLimitSpecify=on  LowerLimitBound=g1_limits(6,1)  LowerLimitBoundUnits=rad  LowerLimitStiffness=g1_stop_k  LowerLimitStiffnessUnits=N*m/rad  LowerLimitDamping=g1_stop_d  LowerLimitDampingUnits=N*m/(rad/s)  LowerLimitTransitionRegionWidth=g1_stop_width  LowerLimitTransitionRegionWidthUnits=rad  UpperLimitSpecify=on  UpperLimitBound=g1_limits(6,2)  UpperLimitBoundUnits=rad  UpperLimitStiffness=g1_stop_k  UpperLimitStiffnessUnits=N*m/rad  UpperLimitDamping=g1_stop_d  UpperLimitDampingUnits=N*m/(rad/s)  UpperLimitTransitionRegionWidth=g1_stop_width  UpperLimitTransitionRegionWidthUnits=rad  TorqueActuationMode=InputTorque  MotionActuationMode=ComputedMotion  SensePosition=on  SenseVelocity=on  SenseAcceleration=off  SenseTorqueForce=off  SenseLowerLimitTorqueForce=off  SenseUpperLimitTorqueForce=off
  left_hip_yaw_link : Subsystem
  left_knee_joint : sm_lib/Joints/Revolute Joint  JointMode=Normal  CompositeWrenchDir=FollowerOnBase  CompositeWrenchFrame=BaseFrame  SenseConstraintForce=off  SenseConstraintTorque=off  SenseTotalForce=off  SenseTotalTorque=off  PositionTargetSpecify=on  PositionTargetPriority=High  PositionTargetValue=g1_q0(7)  PositionTargetValueUnits=rad  VelocityTargetSpecify=on  VelocityTargetPriority=High  VelocityTargetValue=g1_qd0(7)  VelocityTargetValueUnits=rad/s  EquilibriumPosition=0  EquilibriumPositionUnits=deg  SpringStiffness=0  SpringStiffnessUnits=N*m/rad  DampingCoefficient=g1_damping  DampingCoefficientUnits=N*m/(rad/s)  LowerLimitSpecify=on  LowerLimitBound=g1_limits(7,1)  LowerLimitBoundUnits=rad  LowerLimitStiffness=g1_stop_k  LowerLimitStiffnessUnits=N*m/rad  LowerLimitDamping=g1_stop_d  LowerLimitDampingUnits=N*m/(rad/s)  LowerLimitTransitionRegionWidth=g1_stop_width  LowerLimitTransitionRegionWidthUnits=rad  UpperLimitSpecify=on  UpperLimitBound=g1_limits(7,2)  UpperLimitBoundUnits=rad  UpperLimitStiffness=g1_stop_k  UpperLimitStiffnessUnits=N*m/rad  UpperLimitDamping=g1_stop_d  UpperLimitDampingUnits=N*m/(rad/s)  UpperLimitTransitionRegionWidth=g1_stop_width  UpperLimitTransitionRegionWidthUnits=rad  TorqueActuationMode=InputTorque  MotionActuationMode=ComputedMotion  SensePosition=on  SenseVelocity=on  SenseAcceleration=off  SenseTorqueForce=off  SenseLowerLimitTorqueForce=off  SenseUpperLimitTorqueForce=off
  left_knee_link : Subsystem
  left_rubber_hand : Subsystem
  left_rubber_hand_Sensor : sm_lib/Frames and Transforms/Transform Sensor  MeasurementFrame=World  RotationSequence=XYX  SenseAngle=off  SenseAxis=off  SenseQ=off  SenseR=on  SenseRotationSequence=off  SenseOmegaX=off  SenseOmegaY=off  SenseOmegaZ=off  SenseOmega=on  SenseQDot=off  SenseRDot=off  SenseRotationSequenceDot=off  SenseAlphaX=off  SenseAlphaY=off  SenseAlphaZ=off  SenseAlpha=off  SenseQDDot=off  SenseRDDot=off  SenseX=off  SenseY=off  SenseZ=off  SenseXYZ=on  SenseRad=off  SenseAzim=off  SenseDist=off  SenseInc=off  SenseXDot=off  SenseYDot=off  SenseZDot=off  SenseXYZDot=on  SenseRadDot=off  SenseAzimDot=off  SenseDistDot=off  SenseIncDot=off  SenseXDDot=off  SenseYDDot=off  SenseZDDot=off  SenseXYZDDot=off  SenseRadDDot=off  SenseAzimDDot=off  SenseDistDDot=off  SenseIncDDot=off
  left_shoulder_pitch_joint : sm_lib/Joints/Revolute Joint  JointMode=Normal  CompositeWrenchDir=FollowerOnBase  CompositeWrenchFrame=BaseFrame  SenseConstraintForce=off  SenseConstraintTorque=off  SenseTotalForce=off  SenseTotalTorque=off  PositionTargetSpecify=on  PositionTargetPriority=High  PositionTargetValue=g1_q0(8)  PositionTargetValueUnits=rad  VelocityTargetSpecify=on  VelocityTargetPriority=High  VelocityTargetValue=g1_qd0(8)  VelocityTargetValueUnits=rad/s  EquilibriumPosition=0  EquilibriumPositionUnits=deg  SpringStiffness=0  SpringStiffnessUnits=N*m/rad  DampingCoefficient=g1_damping  DampingCoefficientUnits=N*m/(rad/s)  LowerLimitSpecify=on  LowerLimitBound=g1_limits(8,1)  LowerLimitBoundUnits=rad  LowerLimitStiffness=g1_stop_k  LowerLimitStiffnessUnits=N*m/rad  LowerLimitDamping=g1_stop_d  LowerLimitDampingUnits=N*m/(rad/s)  LowerLimitTransitionRegionWidth=g1_stop_width  LowerLimitTransitionRegionWidthUnits=rad  UpperLimitSpecify=on  UpperLimitBound=g1_limits(8,2)  UpperLimitBoundUnits=rad  UpperLimitStiffness=g1_stop_k  UpperLimitStiffnessUnits=N*m/rad  UpperLimitDamping=g1_stop_d  UpperLimitDampingUnits=N*m/(rad/s)  UpperLimitTransitionRegionWidth=g1_stop_width  UpperLimitTransitionRegionWidthUnits=rad  TorqueActuationMode=InputTorque  MotionActuationMode=ComputedMotion  SensePosition=on  SenseVelocity=on  SenseAcceleration=off  SenseTorqueForce=off  SenseLowerLimitTorqueForce=off  SenseUpperLimitTorqueForce=off
  left_shoulder_pitch_link : Subsystem
  left_shoulder_roll_joint : sm_lib/Joints/Revolute Joint  JointMode=Normal  CompositeWrenchDir=FollowerOnBase  CompositeWrenchFrame=BaseFrame  SenseConstraintForce=off  SenseConstraintTorque=off  SenseTotalForce=off  SenseTotalTorque=off  PositionTargetSpecify=on  PositionTargetPriority=High  PositionTargetValue=g1_q0(9)  PositionTargetValueUnits=rad  VelocityTargetSpecify=on  VelocityTargetPriority=High  VelocityTargetValue=g1_qd0(9)  VelocityTargetValueUnits=rad/s  EquilibriumPosition=0  EquilibriumPositionUnits=deg  SpringStiffness=0  SpringStiffnessUnits=N*m/rad  DampingCoefficient=g1_damping  DampingCoefficientUnits=N*m/(rad/s)  LowerLimitSpecify=on  LowerLimitBound=g1_limits(9,1)  LowerLimitBoundUnits=rad  LowerLimitStiffness=g1_stop_k  LowerLimitStiffnessUnits=N*m/rad  LowerLimitDamping=g1_stop_d  LowerLimitDampingUnits=N*m/(rad/s)  LowerLimitTransitionRegionWidth=g1_stop_width  LowerLimitTransitionRegionWidthUnits=rad  UpperLimitSpecify=on  UpperLimitBound=g1_limits(9,2)  UpperLimitBoundUnits=rad  UpperLimitStiffness=g1_stop_k  UpperLimitStiffnessUnits=N*m/rad  UpperLimitDamping=g1_stop_d  UpperLimitDampingUnits=N*m/(rad/s)  UpperLimitTransitionRegionWidth=g1_stop_width  UpperLimitTransitionRegionWidthUnits=rad  TorqueActuationMode=InputTorque  MotionActuationMode=ComputedMotion  SensePosition=on  SenseVelocity=on  SenseAcceleration=off  SenseTorqueForce=off  SenseLowerLimitTorqueForce=off  SenseUpperLimitTorqueForce=off
  left_shoulder_roll_link : Subsystem
  left_shoulder_yaw_joint : sm_lib/Joints/Revolute Joint  JointMode=Normal  CompositeWrenchDir=FollowerOnBase  CompositeWrenchFrame=BaseFrame  SenseConstraintForce=off  SenseConstraintTorque=off  SenseTotalForce=off  SenseTotalTorque=off  PositionTargetSpecify=on  PositionTargetPriority=High  PositionTargetValue=g1_q0(10)  PositionTargetValueUnits=rad  VelocityTargetSpecify=on  VelocityTargetPriority=High  VelocityTargetValue=g1_qd0(10)  VelocityTargetValueUnits=rad/s  EquilibriumPosition=0  EquilibriumPositionUnits=deg  SpringStiffness=0  SpringStiffnessUnits=N*m/rad  DampingCoefficient=g1_damping  DampingCoefficientUnits=N*m/(rad/s)  LowerLimitSpecify=on  LowerLimitBound=g1_limits(10,1)  LowerLimitBoundUnits=rad  LowerLimitStiffness=g1_stop_k  LowerLimitStiffnessUnits=N*m/rad  LowerLimitDamping=g1_stop_d  LowerLimitDampingUnits=N*m/(rad/s)  LowerLimitTransitionRegionWidth=g1_stop_width  LowerLimitTransitionRegionWidthUnits=rad  UpperLimitSpecify=on  UpperLimitBound=g1_limits(10,2)  UpperLimitBoundUnits=rad  UpperLimitStiffness=g1_stop_k  UpperLimitStiffnessUnits=N*m/rad  UpperLimitDamping=g1_stop_d  UpperLimitDampingUnits=N*m/(rad/s)  UpperLimitTransitionRegionWidth=g1_stop_width  UpperLimitTransitionRegionWidthUnits=rad  TorqueActuationMode=InputTorque  MotionActuationMode=ComputedMotion  SensePosition=on  SenseVelocity=on  SenseAcceleration=off  SenseTorqueForce=off  SenseLowerLimitTorqueForce=off  SenseUpperLimitTorqueForce=off
  left_shoulder_yaw_link : Subsystem
  left_wrist_pitch_joint : sm_lib/Joints/Revolute Joint  JointMode=Normal  CompositeWrenchDir=FollowerOnBase  CompositeWrenchFrame=BaseFrame  SenseConstraintForce=off  SenseConstraintTorque=off  SenseTotalForce=off  SenseTotalTorque=off  PositionTargetSpecify=on  PositionTargetPriority=High  PositionTargetValue=g1_q0(11)  PositionTargetValueUnits=rad  VelocityTargetSpecify=on  VelocityTargetPriority=High  VelocityTargetValue=g1_qd0(11)  VelocityTargetValueUnits=rad/s  EquilibriumPosition=0  EquilibriumPositionUnits=deg  SpringStiffness=0  SpringStiffnessUnits=N*m/rad  DampingCoefficient=g1_damping  DampingCoefficientUnits=N*m/(rad/s)  LowerLimitSpecify=on  LowerLimitBound=g1_limits(11,1)  LowerLimitBoundUnits=rad  LowerLimitStiffness=g1_stop_k  LowerLimitStiffnessUnits=N*m/rad  LowerLimitDamping=g1_stop_d  LowerLimitDampingUnits=N*m/(rad/s)  LowerLimitTransitionRegionWidth=g1_stop_width  LowerLimitTransitionRegionWidthUnits=rad  UpperLimitSpecify=on  UpperLimitBound=g1_limits(11,2)  UpperLimitBoundUnits=rad  UpperLimitStiffness=g1_stop_k  UpperLimitStiffnessUnits=N*m/rad  UpperLimitDamping=g1_stop_d  UpperLimitDampingUnits=N*m/(rad/s)  UpperLimitTransitionRegionWidth=g1_stop_width  UpperLimitTransitionRegionWidthUnits=rad  TorqueActuationMode=InputTorque  MotionActuationMode=ComputedMotion  SensePosition=on  SenseVelocity=on  SenseAcceleration=off  SenseTorqueForce=off  SenseLowerLimitTorqueForce=off  SenseUpperLimitTorqueForce=off
  left_wrist_pitch_link : Subsystem
  left_wrist_roll_joint : sm_lib/Joints/Revolute Joint  JointMode=Normal  CompositeWrenchDir=FollowerOnBase  CompositeWrenchFrame=BaseFrame  SenseConstraintForce=off  SenseConstraintTorque=off  SenseTotalForce=off  SenseTotalTorque=off  PositionTargetSpecify=on  PositionTargetPriority=High  PositionTargetValue=g1_q0(12)  PositionTargetValueUnits=rad  VelocityTargetSpecify=on  VelocityTargetPriority=High  VelocityTargetValue=g1_qd0(12)  VelocityTargetValueUnits=rad/s  EquilibriumPosition=0  EquilibriumPositionUnits=deg  SpringStiffness=0  SpringStiffnessUnits=N*m/rad  DampingCoefficient=g1_damping  DampingCoefficientUnits=N*m/(rad/s)  LowerLimitSpecify=on  LowerLimitBound=g1_limits(12,1)  LowerLimitBoundUnits=rad  LowerLimitStiffness=g1_stop_k  LowerLimitStiffnessUnits=N*m/rad  LowerLimitDamping=g1_stop_d  LowerLimitDampingUnits=N*m/(rad/s)  LowerLimitTransitionRegionWidth=g1_stop_width  LowerLimitTransitionRegionWidthUnits=rad  UpperLimitSpecify=on  UpperLimitBound=g1_limits(12,2)  UpperLimitBoundUnits=rad  UpperLimitStiffness=g1_stop_k  UpperLimitStiffnessUnits=N*m/rad  UpperLimitDamping=g1_stop_d  UpperLimitDampingUnits=N*m/(rad/s)  UpperLimitTransitionRegionWidth=g1_stop_width  UpperLimitTransitionRegionWidthUnits=rad  TorqueActuationMode=InputTorque  MotionActuationMode=ComputedMotion  SensePosition=on  SenseVelocity=on  SenseAcceleration=off  SenseTorqueForce=off  SenseLowerLimitTorqueForce=off  SenseUpperLimitTorqueForce=off
  left_wrist_roll_link : Subsystem
  left_wrist_yaw_joint : sm_lib/Joints/Revolute Joint  JointMode=Normal  CompositeWrenchDir=FollowerOnBase  CompositeWrenchFrame=BaseFrame  SenseConstraintForce=off  SenseConstraintTorque=off  SenseTotalForce=off  SenseTotalTorque=off  PositionTargetSpecify=on  PositionTargetPriority=High  PositionTargetValue=g1_q0(13)  PositionTargetValueUnits=rad  VelocityTargetSpecify=on  VelocityTargetPriority=High  VelocityTargetValue=g1_qd0(13)  VelocityTargetValueUnits=rad/s  EquilibriumPosition=0  EquilibriumPositionUnits=deg  SpringStiffness=0  SpringStiffnessUnits=N*m/rad  DampingCoefficient=g1_damping  DampingCoefficientUnits=N*m/(rad/s)  LowerLimitSpecify=on  LowerLimitBound=g1_limits(13,1)  LowerLimitBoundUnits=rad  LowerLimitStiffness=g1_stop_k  LowerLimitStiffnessUnits=N*m/rad  LowerLimitDamping=g1_stop_d  LowerLimitDampingUnits=N*m/(rad/s)  LowerLimitTransitionRegionWidth=g1_stop_width  LowerLimitTransitionRegionWidthUnits=rad  UpperLimitSpecify=on  UpperLimitBound=g1_limits(13,2)  UpperLimitBoundUnits=rad  UpperLimitStiffness=g1_stop_k  UpperLimitStiffnessUnits=N*m/rad  UpperLimitDamping=g1_stop_d  UpperLimitDampingUnits=N*m/(rad/s)  UpperLimitTransitionRegionWidth=g1_stop_width  UpperLimitTransitionRegionWidthUnits=rad  TorqueActuationMode=InputTorque  MotionActuationMode=ComputedMotion  SensePosition=on  SenseVelocity=on  SenseAcceleration=off  SenseTorqueForce=off  SenseLowerLimitTorqueForce=off  SenseUpperLimitTorqueForce=off
  left_wrist_yaw_link : Subsystem
  logo_joint : sm_lib/Joints/Weld Joint  JointMode=Normal  CompositeWrenchDir=FollowerOnBase  CompositeWrenchFrame=BaseFrame  SenseConstraintForce=off  SenseConstraintTorque=off  SenseTotalForce=off  SenseTotalTorque=off
  logo_link : Subsystem
  mid360_joint : sm_lib/Joints/Weld Joint  JointMode=Normal  CompositeWrenchDir=FollowerOnBase  CompositeWrenchFrame=BaseFrame  SenseConstraintForce=off  SenseConstraintTorque=off  SenseTotalForce=off  SenseTotalTorque=off
  mid360_link : Subsystem
  pelvis : Subsystem
  pelvis_Sensor : sm_lib/Frames and Transforms/Transform Sensor  MeasurementFrame=World  RotationSequence=XYX  SenseAngle=off  SenseAxis=off  SenseQ=off  SenseR=on  SenseRotationSequence=off  SenseOmegaX=off  SenseOmegaY=off  SenseOmegaZ=off  SenseOmega=on  SenseQDot=off  SenseRDot=off  SenseRotationSequenceDot=off  SenseAlphaX=off  SenseAlphaY=off  SenseAlphaZ=off  SenseAlpha=off  SenseQDDot=off  SenseRDDot=off  SenseX=off  SenseY=off  SenseZ=off  SenseXYZ=on  SenseRad=off  SenseAzim=off  SenseDist=off  SenseInc=off  SenseXDot=off  SenseYDot=off  SenseZDot=off  SenseXYZDot=on  SenseRadDot=off  SenseAzimDot=off  SenseDistDot=off  SenseIncDot=off  SenseXDDot=off  SenseYDDot=off  SenseZDDot=off  SenseXYZDDot=off  SenseRadDDot=off  SenseAzimDDot=off  SenseDistDDot=off  SenseIncDDot=off
  pelvis_contour_joint : sm_lib/Joints/Weld Joint  JointMode=Normal  CompositeWrenchDir=FollowerOnBase  CompositeWrenchFrame=BaseFrame  SenseConstraintForce=off  SenseConstraintTorque=off  SenseTotalForce=off  SenseTotalTorque=off
  pelvis_contour_link : Subsystem
  right_ankle_pitch_joint : sm_lib/Joints/Revolute Joint  JointMode=Normal  CompositeWrenchDir=FollowerOnBase  CompositeWrenchFrame=BaseFrame  SenseConstraintForce=off  SenseConstraintTorque=off  SenseTotalForce=off  SenseTotalTorque=off  PositionTargetSpecify=on  PositionTargetPriority=High  PositionTargetValue=g1_q0(14)  PositionTargetValueUnits=rad  VelocityTargetSpecify=on  VelocityTargetPriority=High  VelocityTargetValue=g1_qd0(14)  VelocityTargetValueUnits=rad/s  EquilibriumPosition=0  EquilibriumPositionUnits=deg  SpringStiffness=0  SpringStiffnessUnits=N*m/rad  DampingCoefficient=g1_damping  DampingCoefficientUnits=N*m/(rad/s)  LowerLimitSpecify=on  LowerLimitBound=g1_limits(14,1)  LowerLimitBoundUnits=rad  LowerLimitStiffness=g1_stop_k  LowerLimitStiffnessUnits=N*m/rad  LowerLimitDamping=g1_stop_d  LowerLimitDampingUnits=N*m/(rad/s)  LowerLimitTransitionRegionWidth=g1_stop_width  LowerLimitTransitionRegionWidthUnits=rad  UpperLimitSpecify=on  UpperLimitBound=g1_limits(14,2)  UpperLimitBoundUnits=rad  UpperLimitStiffness=g1_stop_k  UpperLimitStiffnessUnits=N*m/rad  UpperLimitDamping=g1_stop_d  UpperLimitDampingUnits=N*m/(rad/s)  UpperLimitTransitionRegionWidth=g1_stop_width  UpperLimitTransitionRegionWidthUnits=rad  TorqueActuationMode=InputTorque  MotionActuationMode=ComputedMotion  SensePosition=on  SenseVelocity=on  SenseAcceleration=off  SenseTorqueForce=off  SenseLowerLimitTorqueForce=off  SenseUpperLimitTorqueForce=off
  right_ankle_pitch_link : Subsystem
  right_ankle_roll_joint : sm_lib/Joints/Revolute Joint  JointMode=Normal  CompositeWrenchDir=FollowerOnBase  CompositeWrenchFrame=BaseFrame  SenseConstraintForce=off  SenseConstraintTorque=off  SenseTotalForce=off  SenseTotalTorque=off  PositionTargetSpecify=on  PositionTargetPriority=High  PositionTargetValue=g1_q0(15)  PositionTargetValueUnits=rad  VelocityTargetSpecify=on  VelocityTargetPriority=High  VelocityTargetValue=g1_qd0(15)  VelocityTargetValueUnits=rad/s  EquilibriumPosition=0  EquilibriumPositionUnits=deg  SpringStiffness=0  SpringStiffnessUnits=N*m/rad  DampingCoefficient=g1_damping  DampingCoefficientUnits=N*m/(rad/s)  LowerLimitSpecify=on  LowerLimitBound=g1_limits(15,1)  LowerLimitBoundUnits=rad  LowerLimitStiffness=g1_stop_k  LowerLimitStiffnessUnits=N*m/rad  LowerLimitDamping=g1_stop_d  LowerLimitDampingUnits=N*m/(rad/s)  LowerLimitTransitionRegionWidth=g1_stop_width  LowerLimitTransitionRegionWidthUnits=rad  UpperLimitSpecify=on  UpperLimitBound=g1_limits(15,2)  UpperLimitBoundUnits=rad  UpperLimitStiffness=g1_stop_k  UpperLimitStiffnessUnits=N*m/rad  UpperLimitDamping=g1_stop_d  UpperLimitDampingUnits=N*m/(rad/s)  UpperLimitTransitionRegionWidth=g1_stop_width  UpperLimitTransitionRegionWidthUnits=rad  TorqueActuationMode=InputTorque  MotionActuationMode=ComputedMotion  SensePosition=on  SenseVelocity=on  SenseAcceleration=off  SenseTorqueForce=off  SenseLowerLimitTorqueForce=off  SenseUpperLimitTorqueForce=off
  right_ankle_roll_link : Subsystem
  right_elbow_joint : sm_lib/Joints/Revolute Joint  JointMode=Normal  CompositeWrenchDir=FollowerOnBase  CompositeWrenchFrame=BaseFrame  SenseConstraintForce=off  SenseConstraintTorque=off  SenseTotalForce=off  SenseTotalTorque=off  PositionTargetSpecify=on  PositionTargetPriority=High  PositionTargetValue=g1_q0(16)  PositionTargetValueUnits=rad  VelocityTargetSpecify=on  VelocityTargetPriority=High  VelocityTargetValue=g1_qd0(16)  VelocityTargetValueUnits=rad/s  EquilibriumPosition=0  EquilibriumPositionUnits=deg  SpringStiffness=0  SpringStiffnessUnits=N*m/rad  DampingCoefficient=g1_damping  DampingCoefficientUnits=N*m/(rad/s)  LowerLimitSpecify=on  LowerLimitBound=g1_limits(16,1)  LowerLimitBoundUnits=rad  LowerLimitStiffness=g1_stop_k  LowerLimitStiffnessUnits=N*m/rad  LowerLimitDamping=g1_stop_d  LowerLimitDampingUnits=N*m/(rad/s)  LowerLimitTransitionRegionWidth=g1_stop_width  LowerLimitTransitionRegionWidthUnits=rad  UpperLimitSpecify=on  UpperLimitBound=g1_limits(16,2)  UpperLimitBoundUnits=rad  UpperLimitStiffness=g1_stop_k  UpperLimitStiffnessUnits=N*m/rad  UpperLimitDamping=g1_stop_d  UpperLimitDampingUnits=N*m/(rad/s)  UpperLimitTransitionRegionWidth=g1_stop_width  UpperLimitTransitionRegionWidthUnits=rad  TorqueActuationMode=InputTorque  MotionActuationMode=ComputedMotion  SensePosition=on  SenseVelocity=on  SenseAcceleration=off  SenseTorqueForce=off  SenseLowerLimitTorqueForce=off  SenseUpperLimitTorqueForce=off
  right_elbow_link : Subsystem
  right_hand_palm_joint : sm_lib/Joints/Weld Joint  JointMode=Normal  CompositeWrenchDir=FollowerOnBase  CompositeWrenchFrame=BaseFrame  SenseConstraintForce=off  SenseConstraintTorque=off  SenseTotalForce=off  SenseTotalTorque=off
  right_hip_pitch_joint : sm_lib/Joints/Revolute Joint  JointMode=Normal  CompositeWrenchDir=FollowerOnBase  CompositeWrenchFrame=BaseFrame  SenseConstraintForce=off  SenseConstraintTorque=off  SenseTotalForce=off  SenseTotalTorque=off  PositionTargetSpecify=on  PositionTargetPriority=High  PositionTargetValue=g1_q0(17)  PositionTargetValueUnits=rad  VelocityTargetSpecify=on  VelocityTargetPriority=High  VelocityTargetValue=g1_qd0(17)  VelocityTargetValueUnits=rad/s  EquilibriumPosition=0  EquilibriumPositionUnits=deg  SpringStiffness=0  SpringStiffnessUnits=N*m/rad  DampingCoefficient=g1_damping  DampingCoefficientUnits=N*m/(rad/s)  LowerLimitSpecify=on  LowerLimitBound=g1_limits(17,1)  LowerLimitBoundUnits=rad  LowerLimitStiffness=g1_stop_k  LowerLimitStiffnessUnits=N*m/rad  LowerLimitDamping=g1_stop_d  LowerLimitDampingUnits=N*m/(rad/s)  LowerLimitTransitionRegionWidth=g1_stop_width  LowerLimitTransitionRegionWidthUnits=rad  UpperLimitSpecify=on  UpperLimitBound=g1_limits(17,2)  UpperLimitBoundUnits=rad  UpperLimitStiffness=g1_stop_k  UpperLimitStiffnessUnits=N*m/rad  UpperLimitDamping=g1_stop_d  UpperLimitDampingUnits=N*m/(rad/s)  UpperLimitTransitionRegionWidth=g1_stop_width  UpperLimitTransitionRegionWidthUnits=rad  TorqueActuationMode=InputTorque  MotionActuationMode=ComputedMotion  SensePosition=on  SenseVelocity=on  SenseAcceleration=off  SenseTorqueForce=off  SenseLowerLimitTorqueForce=off  SenseUpperLimitTorqueForce=off
  right_hip_pitch_link : Subsystem
  right_hip_roll_joint : sm_lib/Joints/Revolute Joint  JointMode=Normal  CompositeWrenchDir=FollowerOnBase  CompositeWrenchFrame=BaseFrame  SenseConstraintForce=off  SenseConstraintTorque=off  SenseTotalForce=off  SenseTotalTorque=off  PositionTargetSpecify=on  PositionTargetPriority=High  PositionTargetValue=g1_q0(18)  PositionTargetValueUnits=rad  VelocityTargetSpecify=on  VelocityTargetPriority=High  VelocityTargetValue=g1_qd0(18)  VelocityTargetValueUnits=rad/s  EquilibriumPosition=0  EquilibriumPositionUnits=deg  SpringStiffness=0  SpringStiffnessUnits=N*m/rad  DampingCoefficient=g1_damping  DampingCoefficientUnits=N*m/(rad/s)  LowerLimitSpecify=on  LowerLimitBound=g1_limits(18,1)  LowerLimitBoundUnits=rad  LowerLimitStiffness=g1_stop_k  LowerLimitStiffnessUnits=N*m/rad  LowerLimitDamping=g1_stop_d  LowerLimitDampingUnits=N*m/(rad/s)  LowerLimitTransitionRegionWidth=g1_stop_width  LowerLimitTransitionRegionWidthUnits=rad  UpperLimitSpecify=on  UpperLimitBound=g1_limits(18,2)  UpperLimitBoundUnits=rad  UpperLimitStiffness=g1_stop_k  UpperLimitStiffnessUnits=N*m/rad  UpperLimitDamping=g1_stop_d  UpperLimitDampingUnits=N*m/(rad/s)  UpperLimitTransitionRegionWidth=g1_stop_width  UpperLimitTransitionRegionWidthUnits=rad  TorqueActuationMode=InputTorque  MotionActuationMode=ComputedMotion  SensePosition=on  SenseVelocity=on  SenseAcceleration=off  SenseTorqueForce=off  SenseLowerLimitTorqueForce=off  SenseUpperLimitTorqueForce=off
  right_hip_roll_link : Subsystem
  right_hip_yaw_joint : sm_lib/Joints/Revolute Joint  JointMode=Normal  CompositeWrenchDir=FollowerOnBase  CompositeWrenchFrame=BaseFrame  SenseConstraintForce=off  SenseConstraintTorque=off  SenseTotalForce=off  SenseTotalTorque=off  PositionTargetSpecify=on  PositionTargetPriority=High  PositionTargetValue=g1_q0(19)  PositionTargetValueUnits=rad  VelocityTargetSpecify=on  VelocityTargetPriority=High  VelocityTargetValue=g1_qd0(19)  VelocityTargetValueUnits=rad/s  EquilibriumPosition=0  EquilibriumPositionUnits=deg  SpringStiffness=0  SpringStiffnessUnits=N*m/rad  DampingCoefficient=g1_damping  DampingCoefficientUnits=N*m/(rad/s)  LowerLimitSpecify=on  LowerLimitBound=g1_limits(19,1)  LowerLimitBoundUnits=rad  LowerLimitStiffness=g1_stop_k  LowerLimitStiffnessUnits=N*m/rad  LowerLimitDamping=g1_stop_d  LowerLimitDampingUnits=N*m/(rad/s)  LowerLimitTransitionRegionWidth=g1_stop_width  LowerLimitTransitionRegionWidthUnits=rad  UpperLimitSpecify=on  UpperLimitBound=g1_limits(19,2)  UpperLimitBoundUnits=rad  UpperLimitStiffness=g1_stop_k  UpperLimitStiffnessUnits=N*m/rad  UpperLimitDamping=g1_stop_d  UpperLimitDampingUnits=N*m/(rad/s)  UpperLimitTransitionRegionWidth=g1_stop_width  UpperLimitTransitionRegionWidthUnits=rad  TorqueActuationMode=InputTorque  MotionActuationMode=ComputedMotion  SensePosition=on  SenseVelocity=on  SenseAcceleration=off  SenseTorqueForce=off  SenseLowerLimitTorqueForce=off  SenseUpperLimitTorqueForce=off
  right_hip_yaw_link : Subsystem
  right_knee_joint : sm_lib/Joints/Revolute Joint  JointMode=Normal  CompositeWrenchDir=FollowerOnBase  CompositeWrenchFrame=BaseFrame  SenseConstraintForce=off  SenseConstraintTorque=off  SenseTotalForce=off  SenseTotalTorque=off  PositionTargetSpecify=on  PositionTargetPriority=High  PositionTargetValue=g1_q0(20)  PositionTargetValueUnits=rad  VelocityTargetSpecify=on  VelocityTargetPriority=High  VelocityTargetValue=g1_qd0(20)  VelocityTargetValueUnits=rad/s  EquilibriumPosition=0  EquilibriumPositionUnits=deg  SpringStiffness=0  SpringStiffnessUnits=N*m/rad  DampingCoefficient=g1_damping  DampingCoefficientUnits=N*m/(rad/s)  LowerLimitSpecify=on  LowerLimitBound=g1_limits(20,1)  LowerLimitBoundUnits=rad  LowerLimitStiffness=g1_stop_k  LowerLimitStiffnessUnits=N*m/rad  LowerLimitDamping=g1_stop_d  LowerLimitDampingUnits=N*m/(rad/s)  LowerLimitTransitionRegionWidth=g1_stop_width  LowerLimitTransitionRegionWidthUnits=rad  UpperLimitSpecify=on  UpperLimitBound=g1_limits(20,2)  UpperLimitBoundUnits=rad  UpperLimitStiffness=g1_stop_k  UpperLimitStiffnessUnits=N*m/rad  UpperLimitDamping=g1_stop_d  UpperLimitDampingUnits=N*m/(rad/s)  UpperLimitTransitionRegionWidth=g1_stop_width  UpperLimitTransitionRegionWidthUnits=rad  TorqueActuationMode=InputTorque  MotionActuationMode=ComputedMotion  SensePosition=on  SenseVelocity=on  SenseAcceleration=off  SenseTorqueForce=off  SenseLowerLimitTorqueForce=off  SenseUpperLimitTorqueForce=off
  right_knee_link : Subsystem
  right_rubber_hand : Subsystem
  right_rubber_hand_Sensor : sm_lib/Frames and Transforms/Transform Sensor  MeasurementFrame=World  RotationSequence=XYX  SenseAngle=off  SenseAxis=off  SenseQ=off  SenseR=on  SenseRotationSequence=off  SenseOmegaX=off  SenseOmegaY=off  SenseOmegaZ=off  SenseOmega=on  SenseQDot=off  SenseRDot=off  SenseRotationSequenceDot=off  SenseAlphaX=off  SenseAlphaY=off  SenseAlphaZ=off  SenseAlpha=off  SenseQDDot=off  SenseRDDot=off  SenseX=off  SenseY=off  SenseZ=off  SenseXYZ=on  SenseRad=off  SenseAzim=off  SenseDist=off  SenseInc=off  SenseXDot=off  SenseYDot=off  SenseZDot=off  SenseXYZDot=on  SenseRadDot=off  SenseAzimDot=off  SenseDistDot=off  SenseIncDot=off  SenseXDDot=off  SenseYDDot=off  SenseZDDot=off  SenseXYZDDot=off  SenseRadDDot=off  SenseAzimDDot=off  SenseDistDDot=off  SenseIncDDot=off
  right_shoulder_pitch_joint : sm_lib/Joints/Revolute Joint  JointMode=Normal  CompositeWrenchDir=FollowerOnBase  CompositeWrenchFrame=BaseFrame  SenseConstraintForce=off  SenseConstraintTorque=off  SenseTotalForce=off  SenseTotalTorque=off  PositionTargetSpecify=on  PositionTargetPriority=High  PositionTargetValue=g1_q0(21)  PositionTargetValueUnits=rad  VelocityTargetSpecify=on  VelocityTargetPriority=High  VelocityTargetValue=g1_qd0(21)  VelocityTargetValueUnits=rad/s  EquilibriumPosition=0  EquilibriumPositionUnits=deg  SpringStiffness=0  SpringStiffnessUnits=N*m/rad  DampingCoefficient=g1_damping  DampingCoefficientUnits=N*m/(rad/s)  LowerLimitSpecify=on  LowerLimitBound=g1_limits(21,1)  LowerLimitBoundUnits=rad  LowerLimitStiffness=g1_stop_k  LowerLimitStiffnessUnits=N*m/rad  LowerLimitDamping=g1_stop_d  LowerLimitDampingUnits=N*m/(rad/s)  LowerLimitTransitionRegionWidth=g1_stop_width  LowerLimitTransitionRegionWidthUnits=rad  UpperLimitSpecify=on  UpperLimitBound=g1_limits(21,2)  UpperLimitBoundUnits=rad  UpperLimitStiffness=g1_stop_k  UpperLimitStiffnessUnits=N*m/rad  UpperLimitDamping=g1_stop_d  UpperLimitDampingUnits=N*m/(rad/s)  UpperLimitTransitionRegionWidth=g1_stop_width  UpperLimitTransitionRegionWidthUnits=rad  TorqueActuationMode=InputTorque  MotionActuationMode=ComputedMotion  SensePosition=on  SenseVelocity=on  SenseAcceleration=off  SenseTorqueForce=off  SenseLowerLimitTorqueForce=off  SenseUpperLimitTorqueForce=off
  right_shoulder_pitch_link : Subsystem
  right_shoulder_roll_joint : sm_lib/Joints/Revolute Joint  JointMode=Normal  CompositeWrenchDir=FollowerOnBase  CompositeWrenchFrame=BaseFrame  SenseConstraintForce=off  SenseConstraintTorque=off  SenseTotalForce=off  SenseTotalTorque=off  PositionTargetSpecify=on  PositionTargetPriority=High  PositionTargetValue=g1_q0(22)  PositionTargetValueUnits=rad  VelocityTargetSpecify=on  VelocityTargetPriority=High  VelocityTargetValue=g1_qd0(22)  VelocityTargetValueUnits=rad/s  EquilibriumPosition=0  EquilibriumPositionUnits=deg  SpringStiffness=0  SpringStiffnessUnits=N*m/rad  DampingCoefficient=g1_damping  DampingCoefficientUnits=N*m/(rad/s)  LowerLimitSpecify=on  LowerLimitBound=g1_limits(22,1)  LowerLimitBoundUnits=rad  LowerLimitStiffness=g1_stop_k  LowerLimitStiffnessUnits=N*m/rad  LowerLimitDamping=g1_stop_d  LowerLimitDampingUnits=N*m/(rad/s)  LowerLimitTransitionRegionWidth=g1_stop_width  LowerLimitTransitionRegionWidthUnits=rad  UpperLimitSpecify=on  UpperLimitBound=g1_limits(22,2)  UpperLimitBoundUnits=rad  UpperLimitStiffness=g1_stop_k  UpperLimitStiffnessUnits=N*m/rad  UpperLimitDamping=g1_stop_d  UpperLimitDampingUnits=N*m/(rad/s)  UpperLimitTransitionRegionWidth=g1_stop_width  UpperLimitTransitionRegionWidthUnits=rad  TorqueActuationMode=InputTorque  MotionActuationMode=ComputedMotion  SensePosition=on  SenseVelocity=on  SenseAcceleration=off  SenseTorqueForce=off  SenseLowerLimitTorqueForce=off  SenseUpperLimitTorqueForce=off
  right_shoulder_roll_link : Subsystem
  right_shoulder_yaw_joint : sm_lib/Joints/Revolute Joint  JointMode=Normal  CompositeWrenchDir=FollowerOnBase  CompositeWrenchFrame=BaseFrame  SenseConstraintForce=off  SenseConstraintTorque=off  SenseTotalForce=off  SenseTotalTorque=off  PositionTargetSpecify=on  PositionTargetPriority=High  PositionTargetValue=g1_q0(23)  PositionTargetValueUnits=rad  VelocityTargetSpecify=on  VelocityTargetPriority=High  VelocityTargetValue=g1_qd0(23)  VelocityTargetValueUnits=rad/s  EquilibriumPosition=0  EquilibriumPositionUnits=deg  SpringStiffness=0  SpringStiffnessUnits=N*m/rad  DampingCoefficient=g1_damping  DampingCoefficientUnits=N*m/(rad/s)  LowerLimitSpecify=on  LowerLimitBound=g1_limits(23,1)  LowerLimitBoundUnits=rad  LowerLimitStiffness=g1_stop_k  LowerLimitStiffnessUnits=N*m/rad  LowerLimitDamping=g1_stop_d  LowerLimitDampingUnits=N*m/(rad/s)  LowerLimitTransitionRegionWidth=g1_stop_width  LowerLimitTransitionRegionWidthUnits=rad  UpperLimitSpecify=on  UpperLimitBound=g1_limits(23,2)  UpperLimitBoundUnits=rad  UpperLimitStiffness=g1_stop_k  UpperLimitStiffnessUnits=N*m/rad  UpperLimitDamping=g1_stop_d  UpperLimitDampingUnits=N*m/(rad/s)  UpperLimitTransitionRegionWidth=g1_stop_width  UpperLimitTransitionRegionWidthUnits=rad  TorqueActuationMode=InputTorque  MotionActuationMode=ComputedMotion  SensePosition=on  SenseVelocity=on  SenseAcceleration=off  SenseTorqueForce=off  SenseLowerLimitTorqueForce=off  SenseUpperLimitTorqueForce=off
  right_shoulder_yaw_link : Subsystem
  right_wrist_pitch_joint : sm_lib/Joints/Revolute Joint  JointMode=Normal  CompositeWrenchDir=FollowerOnBase  CompositeWrenchFrame=BaseFrame  SenseConstraintForce=off  SenseConstraintTorque=off  SenseTotalForce=off  SenseTotalTorque=off  PositionTargetSpecify=on  PositionTargetPriority=High  PositionTargetValue=g1_q0(24)  PositionTargetValueUnits=rad  VelocityTargetSpecify=on  VelocityTargetPriority=High  VelocityTargetValue=g1_qd0(24)  VelocityTargetValueUnits=rad/s  EquilibriumPosition=0  EquilibriumPositionUnits=deg  SpringStiffness=0  SpringStiffnessUnits=N*m/rad  DampingCoefficient=g1_damping  DampingCoefficientUnits=N*m/(rad/s)  LowerLimitSpecify=on  LowerLimitBound=g1_limits(24,1)  LowerLimitBoundUnits=rad  LowerLimitStiffness=g1_stop_k  LowerLimitStiffnessUnits=N*m/rad  LowerLimitDamping=g1_stop_d  LowerLimitDampingUnits=N*m/(rad/s)  LowerLimitTransitionRegionWidth=g1_stop_width  LowerLimitTransitionRegionWidthUnits=rad  UpperLimitSpecify=on  UpperLimitBound=g1_limits(24,2)  UpperLimitBoundUnits=rad  UpperLimitStiffness=g1_stop_k  UpperLimitStiffnessUnits=N*m/rad  UpperLimitDamping=g1_stop_d  UpperLimitDampingUnits=N*m/(rad/s)  UpperLimitTransitionRegionWidth=g1_stop_width  UpperLimitTransitionRegionWidthUnits=rad  TorqueActuationMode=InputTorque  MotionActuationMode=ComputedMotion  SensePosition=on  SenseVelocity=on  SenseAcceleration=off  SenseTorqueForce=off  SenseLowerLimitTorqueForce=off  SenseUpperLimitTorqueForce=off
  right_wrist_pitch_link : Subsystem
  right_wrist_roll_joint : sm_lib/Joints/Revolute Joint  JointMode=Normal  CompositeWrenchDir=FollowerOnBase  CompositeWrenchFrame=BaseFrame  SenseConstraintForce=off  SenseConstraintTorque=off  SenseTotalForce=off  SenseTotalTorque=off  PositionTargetSpecify=on  PositionTargetPriority=High  PositionTargetValue=g1_q0(25)  PositionTargetValueUnits=rad  VelocityTargetSpecify=on  VelocityTargetPriority=High  VelocityTargetValue=g1_qd0(25)  VelocityTargetValueUnits=rad/s  EquilibriumPosition=0  EquilibriumPositionUnits=deg  SpringStiffness=0  SpringStiffnessUnits=N*m/rad  DampingCoefficient=g1_damping  DampingCoefficientUnits=N*m/(rad/s)  LowerLimitSpecify=on  LowerLimitBound=g1_limits(25,1)  LowerLimitBoundUnits=rad  LowerLimitStiffness=g1_stop_k  LowerLimitStiffnessUnits=N*m/rad  LowerLimitDamping=g1_stop_d  LowerLimitDampingUnits=N*m/(rad/s)  LowerLimitTransitionRegionWidth=g1_stop_width  LowerLimitTransitionRegionWidthUnits=rad  UpperLimitSpecify=on  UpperLimitBound=g1_limits(25,2)  UpperLimitBoundUnits=rad  UpperLimitStiffness=g1_stop_k  UpperLimitStiffnessUnits=N*m/rad  UpperLimitDamping=g1_stop_d  UpperLimitDampingUnits=N*m/(rad/s)  UpperLimitTransitionRegionWidth=g1_stop_width  UpperLimitTransitionRegionWidthUnits=rad  TorqueActuationMode=InputTorque  MotionActuationMode=ComputedMotion  SensePosition=on  SenseVelocity=on  SenseAcceleration=off  SenseTorqueForce=off  SenseLowerLimitTorqueForce=off  SenseUpperLimitTorqueForce=off
  right_wrist_roll_link : Subsystem
  right_wrist_yaw_joint : sm_lib/Joints/Revolute Joint  JointMode=Normal  CompositeWrenchDir=FollowerOnBase  CompositeWrenchFrame=BaseFrame  SenseConstraintForce=off  SenseConstraintTorque=off  SenseTotalForce=off  SenseTotalTorque=off  PositionTargetSpecify=on  PositionTargetPriority=High  PositionTargetValue=g1_q0(26)  PositionTargetValueUnits=rad  VelocityTargetSpecify=on  VelocityTargetPriority=High  VelocityTargetValue=g1_qd0(26)  VelocityTargetValueUnits=rad/s  EquilibriumPosition=0  EquilibriumPositionUnits=deg  SpringStiffness=0  SpringStiffnessUnits=N*m/rad  DampingCoefficient=g1_damping  DampingCoefficientUnits=N*m/(rad/s)  LowerLimitSpecify=on  LowerLimitBound=g1_limits(26,1)  LowerLimitBoundUnits=rad  LowerLimitStiffness=g1_stop_k  LowerLimitStiffnessUnits=N*m/rad  LowerLimitDamping=g1_stop_d  LowerLimitDampingUnits=N*m/(rad/s)  LowerLimitTransitionRegionWidth=g1_stop_width  LowerLimitTransitionRegionWidthUnits=rad  UpperLimitSpecify=on  UpperLimitBound=g1_limits(26,2)  UpperLimitBoundUnits=rad  UpperLimitStiffness=g1_stop_k  UpperLimitStiffnessUnits=N*m/rad  UpperLimitDamping=g1_stop_d  UpperLimitDampingUnits=N*m/(rad/s)  UpperLimitTransitionRegionWidth=g1_stop_width  UpperLimitTransitionRegionWidthUnits=rad  TorqueActuationMode=InputTorque  MotionActuationMode=ComputedMotion  SensePosition=on  SenseVelocity=on  SenseAcceleration=off  SenseTorqueForce=off  SenseLowerLimitTorqueForce=off  SenseUpperLimitTorqueForce=off
  right_wrist_yaw_link : Subsystem
  torso_link : Subsystem
  waist_pitch_joint : sm_lib/Joints/Revolute Joint  JointMode=Normal  CompositeWrenchDir=FollowerOnBase  CompositeWrenchFrame=BaseFrame  SenseConstraintForce=off  SenseConstraintTorque=off  SenseTotalForce=off  SenseTotalTorque=off  PositionTargetSpecify=on  PositionTargetPriority=High  PositionTargetValue=g1_q0(27)  PositionTargetValueUnits=rad  VelocityTargetSpecify=on  VelocityTargetPriority=High  VelocityTargetValue=g1_qd0(27)  VelocityTargetValueUnits=rad/s  EquilibriumPosition=0  EquilibriumPositionUnits=deg  SpringStiffness=0  SpringStiffnessUnits=N*m/rad  DampingCoefficient=g1_damping  DampingCoefficientUnits=N*m/(rad/s)  LowerLimitSpecify=on  LowerLimitBound=g1_limits(27,1)  LowerLimitBoundUnits=rad  LowerLimitStiffness=g1_stop_k  LowerLimitStiffnessUnits=N*m/rad  LowerLimitDamping=g1_stop_d  LowerLimitDampingUnits=N*m/(rad/s)  LowerLimitTransitionRegionWidth=g1_stop_width  LowerLimitTransitionRegionWidthUnits=rad  UpperLimitSpecify=on  UpperLimitBound=g1_limits(27,2)  UpperLimitBoundUnits=rad  UpperLimitStiffness=g1_stop_k  UpperLimitStiffnessUnits=N*m/rad  UpperLimitDamping=g1_stop_d  UpperLimitDampingUnits=N*m/(rad/s)  UpperLimitTransitionRegionWidth=g1_stop_width  UpperLimitTransitionRegionWidthUnits=rad  TorqueActuationMode=InputTorque  MotionActuationMode=ComputedMotion  SensePosition=on  SenseVelocity=on  SenseAcceleration=off  SenseTorqueForce=off  SenseLowerLimitTorqueForce=off  SenseUpperLimitTorqueForce=off
  waist_roll_joint : sm_lib/Joints/Revolute Joint  JointMode=Normal  CompositeWrenchDir=FollowerOnBase  CompositeWrenchFrame=BaseFrame  SenseConstraintForce=off  SenseConstraintTorque=off  SenseTotalForce=off  SenseTotalTorque=off  PositionTargetSpecify=on  PositionTargetPriority=High  PositionTargetValue=g1_q0(28)  PositionTargetValueUnits=rad  VelocityTargetSpecify=on  VelocityTargetPriority=High  VelocityTargetValue=g1_qd0(28)  VelocityTargetValueUnits=rad/s  EquilibriumPosition=0  EquilibriumPositionUnits=deg  SpringStiffness=0  SpringStiffnessUnits=N*m/rad  DampingCoefficient=g1_damping  DampingCoefficientUnits=N*m/(rad/s)  LowerLimitSpecify=on  LowerLimitBound=g1_limits(28,1)  LowerLimitBoundUnits=rad  LowerLimitStiffness=g1_stop_k  LowerLimitStiffnessUnits=N*m/rad  LowerLimitDamping=g1_stop_d  LowerLimitDampingUnits=N*m/(rad/s)  LowerLimitTransitionRegionWidth=g1_stop_width  LowerLimitTransitionRegionWidthUnits=rad  UpperLimitSpecify=on  UpperLimitBound=g1_limits(28,2)  UpperLimitBoundUnits=rad  UpperLimitStiffness=g1_stop_k  UpperLimitStiffnessUnits=N*m/rad  UpperLimitDamping=g1_stop_d  UpperLimitDampingUnits=N*m/(rad/s)  UpperLimitTransitionRegionWidth=g1_stop_width  UpperLimitTransitionRegionWidthUnits=rad  TorqueActuationMode=InputTorque  MotionActuationMode=ComputedMotion  SensePosition=on  SenseVelocity=on  SenseAcceleration=off  SenseTorqueForce=off  SenseLowerLimitTorqueForce=off  SenseUpperLimitTorqueForce=off
  waist_roll_link : Subsystem
  waist_support_joint : sm_lib/Joints/Weld Joint  JointMode=Normal  CompositeWrenchDir=FollowerOnBase  CompositeWrenchFrame=BaseFrame  SenseConstraintForce=off  SenseConstraintTorque=off  SenseTotalForce=off  SenseTotalTorque=off
  waist_support_link : Subsystem
  waist_yaw_joint : sm_lib/Joints/Revolute Joint  JointMode=Normal  CompositeWrenchDir=FollowerOnBase  CompositeWrenchFrame=BaseFrame  SenseConstraintForce=off  SenseConstraintTorque=off  SenseTotalForce=off  SenseTotalTorque=off  PositionTargetSpecify=on  PositionTargetPriority=High  PositionTargetValue=g1_q0(29)  PositionTargetValueUnits=rad  VelocityTargetSpecify=on  VelocityTargetPriority=High  VelocityTargetValue=g1_qd0(29)  VelocityTargetValueUnits=rad/s  EquilibriumPosition=0  EquilibriumPositionUnits=deg  SpringStiffness=0  SpringStiffnessUnits=N*m/rad  DampingCoefficient=g1_damping  DampingCoefficientUnits=N*m/(rad/s)  LowerLimitSpecify=on  LowerLimitBound=g1_limits(29,1)  LowerLimitBoundUnits=rad  LowerLimitStiffness=g1_stop_k  LowerLimitStiffnessUnits=N*m/rad  LowerLimitDamping=g1_stop_d  LowerLimitDampingUnits=N*m/(rad/s)  LowerLimitTransitionRegionWidth=g1_stop_width  LowerLimitTransitionRegionWidthUnits=rad  UpperLimitSpecify=on  UpperLimitBound=g1_limits(29,2)  UpperLimitBoundUnits=rad  UpperLimitStiffness=g1_stop_k  UpperLimitStiffnessUnits=N*m/rad  UpperLimitDamping=g1_stop_d  UpperLimitDampingUnits=N*m/(rad/s)  UpperLimitTransitionRegionWidth=g1_stop_width  UpperLimitTransitionRegionWidthUnits=rad  TorqueActuationMode=InputTorque  MotionActuationMode=ComputedMotion  SensePosition=on  SenseVelocity=on  SenseAcceleration=off  SenseTorqueForce=off  SenseLowerLimitTorqueForce=off  SenseUpperLimitTorqueForce=off
  waist_yaw_link : Subsystem
  q : Outport
  qd : Outport  Port=2
  pelvis_p : Outport  Port=3
  pelvis_R : Outport  Port=4
  pelvis_w : Outport  Port=5
  pelvis_v : Outport  Port=6
  foot_l_contact_p : Outport  Port=7
  foot_l_contact_R : Outport  Port=8
  foot_l_contact_w : Outport  Port=9
  foot_l_contact_v : Outport  Port=10
  foot_r_contact_p : Outport  Port=11
  foot_r_contact_R : Outport  Port=12
  foot_r_contact_w : Outport  Port=13
  foot_r_contact_v : Outport  Port=14
  left_rubber_hand_p : Outport  Port=15
  left_rubber_hand_R : Outport  Port=16
  left_rubber_hand_w : Outport  Port=17
  left_rubber_hand_v : Outport  Port=18
  right_rubber_hand_p : Outport  Port=19
  right_rubber_hand_R : Outport  Port=20
  right_rubber_hand_w : Outport  Port=21
  right_rubber_hand_v : Outport  Port=22
  contact1_1 : Outport  Port=23
  contact1_2 : Outport  Port=24
  contact1_3 : Outport  Port=25
  contact1_4 : Outport  Port=26
  contact1_5 : Outport  Port=27
  contact1_6 : Outport  Port=28
  contact1_7 : Outport  Port=29
  contact2_1 : Outport  Port=30
  contact2_2 : Outport  Port=31
  contact2_3 : Outport  Port=32
  contact2_4 : Outport  Port=33
  contact2_5 : Outport  Port=34
  contact2_6 : Outport  Port=35
  contact2_7 : Outport  Port=36
  wires:
  j28_Position/1 -> JointPositions/28
  frame1p/1 -> pelvis_p/1
  frame1R/1 -> pelvis_R/1
  frame1w/1 -> pelvis_w/1
  frame1v/1 -> pelvis_v/1
  frame2p/1 -> foot_l_contact_p/1
  frame2R/1 -> foot_l_contact_R/1
  frame2w/1 -> foot_l_contact_w/1
  frame2v/1 -> foot_l_contact_v/1
  frame3p/1 -> foot_r_contact_p/1
  frame3R/1 -> foot_r_contact_R/1
  frame3w/1 -> foot_r_contact_w/1
  frame3v/1 -> foot_r_contact_v/1
  frame4p/1 -> left_rubber_hand_p/1
  frame4R/1 -> left_rubber_hand_R/1
  frame4w/1 -> left_rubber_hand_w/1
  frame4v/1 -> left_rubber_hand_v/1
  frame5p/1 -> right_rubber_hand_p/1
  frame5R/1 -> right_rubber_hand_R/1
  frame5w/1 -> right_rubber_hand_w/1
  frame5v/1 -> right_rubber_hand_v/1
  tau_test/1 -> TorqueChannels/1
  JointPositions/1 -> q/1
  JointVelocities/1 -> qd/1
  TorqueChannels/1 -> j01_Torque/1
  j01_Position/1 -> JointPositions/1
  j01_Velocity/1 -> JointVelocities/1
  TorqueChannels/2 -> j02_Torque/1
  j02_Position/1 -> JointPositions/2
  j02_Velocity/1 -> JointVelocities/2
  TorqueChannels/3 -> j03_Torque/1
  j03_Position/1 -> JointPositions/3
  j03_Velocity/1 -> JointVelocities/3
  TorqueChannels/4 -> j04_Torque/1
  j04_Position/1 -> JointPositions/4
  j04_Velocity/1 -> JointVelocities/4
  TorqueChannels/5 -> j05_Torque/1
  j05_Position/1 -> JointPositions/5
  j05_Velocity/1 -> JointVelocities/5
  TorqueChannels/6 -> j06_Torque/1
  j06_Position/1 -> JointPositions/6
  j06_Velocity/1 -> JointVelocities/6
  TorqueChannels/7 -> j07_Torque/1
  j07_Position/1 -> JointPositions/7
  j07_Velocity/1 -> JointVelocities/7
  TorqueChannels/8 -> j08_Torque/1
  j08_Position/1 -> JointPositions/8
  j08_Velocity/1 -> JointVelocities/8
  TorqueChannels/9 -> j09_Torque/1
  j09_Position/1 -> JointPositions/9
  j09_Velocity/1 -> JointVelocities/9
  TorqueChannels/10 -> j10_Torque/1
  j10_Position/1 -> JointPositions/10
  j10_Velocity/1 -> JointVelocities/10
  TorqueChannels/11 -> j11_Torque/1
  j11_Position/1 -> JointPositions/11
  j11_Velocity/1 -> JointVelocities/11
  TorqueChannels/12 -> j12_Torque/1
  j12_Position/1 -> JointPositions/12
  TorqueChannels/13 -> j13_Torque/1
  j13_Position/1 -> JointPositions/13
  j13_Velocity/1 -> JointVelocities/13
  TorqueChannels/14 -> j14_Torque/1
  j14_Position/1 -> JointPositions/14
  j14_Velocity/1 -> JointVelocities/14
  TorqueChannels/15 -> j15_Torque/1
  j15_Position/1 -> JointPositions/15
  j15_Velocity/1 -> JointVelocities/15
  TorqueChannels/16 -> j16_Torque/1
  j16_Position/1 -> JointPositions/16
  j16_Velocity/1 -> JointVelocities/16
  TorqueChannels/17 -> j17_Torque/1
  j17_Position/1 -> JointPositions/17
  j17_Velocity/1 -> JointVelocities/17
  TorqueChannels/18 -> j18_Torque/1
  j18_Position/1 -> JointPositions/18
  j18_Velocity/1 -> JointVelocities/18
  TorqueChannels/19 -> j19_Torque/1
  j19_Position/1 -> JointPositions/19
  j19_Velocity/1 -> JointVelocities/19
  TorqueChannels/20 -> j20_Torque/1
  j20_Position/1 -> JointPositions/20
  j20_Velocity/1 -> JointVelocities/20
  TorqueChannels/21 -> j21_Torque/1
  j21_Position/1 -> JointPositions/21
  j21_Velocity/1 -> JointVelocities/21
  TorqueChannels/22 -> j22_Torque/1
  j22_Position/1 -> JointPositions/22
  j22_Velocity/1 -> JointVelocities/22
  TorqueChannels/23 -> j23_Torque/1
  j23_Position/1 -> JointPositions/23
  j23_Velocity/1 -> JointVelocities/23
  TorqueChannels/24 -> j24_Torque/1
  j24_Position/1 -> JointPositions/24
  j24_Velocity/1 -> JointVelocities/24
  TorqueChannels/25 -> j25_Torque/1
  j25_Velocity/1 -> JointVelocities/25
  TorqueChannels/26 -> j26_Torque/1
  j26_Position/1 -> JointPositions/26
  j26_Velocity/1 -> JointVelocities/26
  TorqueChannels/27 -> j27_Torque/1
  j27_Position/1 -> JointPositions/27
  j27_Velocity/1 -> JointVelocities/27
  TorqueChannels/28 -> j28_Torque/1
  j28_Velocity/1 -> JointVelocities/28
  TorqueChannels/29 -> j29_Torque/1
  j29_Position/1 -> JointPositions/29
  j29_Velocity/1 -> JointVelocities/29
  RightFootContact/7(ContactPositionGroundOut) -> contact2_7/1
  RightFootContact/6(SlipVelocityOut) -> contact2_6/1
  RightFootContact/5(PointTotalTorqueOut) -> contact2_5/1
  RightFootContact/4(PointTotalForceOut) -> contact2_4/1
  RightFootContact/3(PointFrictionForceOut) -> contact2_3/1
  RightFootContact/2(PointNormalForceOut) -> contact2_2/1
  RightFootContact/1(PenetrationOut) -> contact2_1/1
  LeftFootContact/7(ContactPositionGroundOut) -> contact1_7/1
  LeftFootContact/6(SlipVelocityOut) -> contact1_6/1
  LeftFootContact/5(PointTotalTorqueOut) -> contact1_5/1
  LeftFootContact/4(PointTotalForceOut) -> contact1_4/1
  LeftFootContact/3(PointFrictionForceOut) -> contact1_3/1
  LeftFootContact/2(PointNormalForceOut) -> contact1_2/1
  LeftFootContact/1(PenetrationOut) -> contact1_1/1
  j25_Position/1 -> JointPositions/25
  j12_Velocity/1 -> JointVelocities/12
  connections:
  FloatingBase/RConn1 -- pelvis/LConn1
  imu_in_pelvis_joint/LConn1 -- pelvis/RConn5
  left_hip_pitch_joint/LConn1 -- pelvis/RConn4
  pelvis/RConn3 -- pelvis_contour_joint/LConn1
  pelvis/RConn2 -- right_hip_pitch_joint/LConn1
  pelvis/RConn1 -- waist_yaw_joint/LConn1
  waist_roll_joint/RConn2 -- j28_Position/LConn1
  pelvis/RConn6 -- pelvis_Sensor/RConn1
  pelvis_Sensor/RConn4 -- frame1p/LConn1
  pelvis_Sensor/RConn2 -- frame1R/LConn1
  pelvis_Sensor/RConn3 -- frame1w/LConn1
  pelvis_Sensor/RConn5 -- frame1v/LConn1
  foot_l_contact_Sensor/RConn4 -- frame2p/LConn1
  foot_l_contact_Sensor/RConn2 -- frame2R/LConn1
  foot_l_contact_Sensor/RConn3 -- frame2w/LConn1
  foot_l_contact_Sensor/RConn5 -- frame2v/LConn1
  foot_r_contact_Sensor/RConn4 -- frame3p/LConn1
  foot_r_contact_Sensor/RConn2 -- frame3R/LConn1
  foot_r_contact_Sensor/RConn3 -- frame3w/LConn1
  foot_r_contact_Sensor/RConn5 -- frame3v/LConn1
  left_rubber_hand/RConn1 -- left_rubber_hand_Sensor/RConn1
  left_rubber_hand_Sensor/RConn4 -- frame4p/LConn1
  left_rubber_hand_Sensor/RConn2 -- frame4R/LConn1
  left_rubber_hand_Sensor/RConn3 -- frame4w/LConn1
  left_rubber_hand_Sensor/RConn5 -- frame4v/LConn1
  right_rubber_hand/RConn1 -- right_rubber_hand_Sensor/RConn1
  right_rubber_hand_Sensor/RConn4 -- frame5p/LConn1
  right_rubber_hand_Sensor/RConn2 -- frame5R/LConn1
  right_rubber_hand_Sensor/RConn3 -- frame5w/LConn1
  right_rubber_hand_Sensor/RConn5 -- frame5v/LConn1
  j01_Torque/RConn1 -- left_ankle_pitch_joint/LConn2
  left_ankle_pitch_joint/RConn2 -- j01_Position/LConn1
  left_ankle_pitch_joint/RConn3 -- j01_Velocity/LConn1
  j02_Torque/RConn1 -- left_ankle_roll_joint/LConn2
  left_ankle_roll_joint/RConn2 -- j02_Position/LConn1
  left_ankle_roll_joint/RConn3 -- j02_Velocity/LConn1
  j03_Torque/RConn1 -- left_elbow_joint/LConn2
  left_elbow_joint/RConn2 -- j03_Position/LConn1
  left_elbow_joint/RConn3 -- j03_Velocity/LConn1
  j04_Torque/RConn1 -- left_hip_pitch_joint/LConn2
  left_hip_pitch_joint/RConn2 -- j04_Position/LConn1
  left_hip_pitch_joint/RConn3 -- j04_Velocity/LConn1
  j05_Torque/RConn1 -- left_hip_roll_joint/LConn2
  left_hip_roll_joint/RConn2 -- j05_Position/LConn1
  left_hip_roll_joint/RConn3 -- j05_Velocity/LConn1
  j06_Torque/RConn1 -- left_hip_yaw_joint/LConn2
  left_hip_yaw_joint/RConn2 -- j06_Position/LConn1
  left_hip_yaw_joint/RConn3 -- j06_Velocity/LConn1
  j07_Torque/RConn1 -- left_knee_joint/LConn2
  left_knee_joint/RConn2 -- j07_Position/LConn1
  left_knee_joint/RConn3 -- j07_Velocity/LConn1
  j08_Torque/RConn1 -- left_shoulder_pitch_joint/LConn2
  left_shoulder_pitch_joint/RConn2 -- j08_Position/LConn1
  left_shoulder_pitch_joint/RConn3 -- j08_Velocity/LConn1
  j09_Torque/RConn1 -- left_shoulder_roll_joint/LConn2
  left_shoulder_roll_joint/RConn2 -- j09_Position/LConn1
  left_shoulder_roll_joint/RConn3 -- j09_Velocity/LConn1
  j10_Torque/RConn1 -- left_shoulder_yaw_joint/LConn2
  left_shoulder_yaw_joint/RConn2 -- j10_Position/LConn1
  left_shoulder_yaw_joint/RConn3 -- j10_Velocity/LConn1
  j11_Torque/RConn1 -- left_wrist_pitch_joint/LConn2
  left_wrist_pitch_joint/RConn2 -- j11_Position/LConn1
  left_wrist_pitch_joint/RConn3 -- j11_Velocity/LConn1
  j12_Torque/RConn1 -- left_wrist_roll_joint/LConn2
  left_wrist_roll_joint/RConn2 -- j12_Position/LConn1
  j13_Torque/RConn1 -- left_wrist_yaw_joint/LConn2
  left_wrist_yaw_joint/RConn2 -- j13_Position/LConn1
  left_wrist_yaw_joint/RConn3 -- j13_Velocity/LConn1
  j14_Torque/RConn1 -- right_ankle_pitch_joint/LConn2
  right_ankle_pitch_joint/RConn2 -- j14_Position/LConn1
  right_ankle_pitch_joint/RConn3 -- j14_Velocity/LConn1
  j15_Torque/RConn1 -- right_ankle_roll_joint/LConn2
  right_ankle_roll_joint/RConn2 -- j15_Position/LConn1
  right_ankle_roll_joint/RConn3 -- j15_Velocity/LConn1
  j16_Torque/RConn1 -- right_elbow_joint/LConn2
  right_elbow_joint/RConn2 -- j16_Position/LConn1
  right_elbow_joint/RConn3 -- j16_Velocity/LConn1
  j17_Torque/RConn1 -- right_hip_pitch_joint/LConn2
  right_hip_pitch_joint/RConn2 -- j17_Position/LConn1
  right_hip_pitch_joint/RConn3 -- j17_Velocity/LConn1
  j18_Torque/RConn1 -- right_hip_roll_joint/LConn2
  right_hip_roll_joint/RConn2 -- j18_Position/LConn1
  right_hip_roll_joint/RConn3 -- j18_Velocity/LConn1
  j19_Torque/RConn1 -- right_hip_yaw_joint/LConn2
  right_hip_yaw_joint/RConn2 -- j19_Position/LConn1
  right_hip_yaw_joint/RConn3 -- j19_Velocity/LConn1
  j20_Torque/RConn1 -- right_knee_joint/LConn2
  right_knee_joint/RConn2 -- j20_Position/LConn1
  right_knee_joint/RConn3 -- j20_Velocity/LConn1
  j21_Torque/RConn1 -- right_shoulder_pitch_joint/LConn2
  right_shoulder_pitch_joint/RConn2 -- j21_Position/LConn1
  right_shoulder_pitch_joint/RConn3 -- j21_Velocity/LConn1
  j22_Torque/RConn1 -- right_shoulder_roll_joint/LConn2
  right_shoulder_roll_joint/RConn2 -- j22_Position/LConn1
  right_shoulder_roll_joint/RConn3 -- j22_Velocity/LConn1
  j23_Torque/RConn1 -- right_shoulder_yaw_joint/LConn2
  right_shoulder_yaw_joint/RConn2 -- j23_Position/LConn1
  right_shoulder_yaw_joint/RConn3 -- j23_Velocity/LConn1
  j24_Torque/RConn1 -- right_wrist_pitch_joint/LConn2
  right_wrist_pitch_joint/RConn2 -- j24_Position/LConn1
  right_wrist_pitch_joint/RConn3 -- j24_Velocity/LConn1
  j25_Torque/RConn1 -- right_wrist_roll_joint/LConn2
  right_wrist_roll_joint/RConn3 -- j25_Velocity/LConn1
  j26_Torque/RConn1 -- right_wrist_yaw_joint/LConn2
  right_wrist_yaw_joint/RConn2 -- j26_Position/LConn1
  right_wrist_yaw_joint/RConn3 -- j26_Velocity/LConn1
  j27_Torque/RConn1 -- waist_pitch_joint/LConn2
  waist_pitch_joint/RConn2 -- j27_Position/LConn1
  waist_pitch_joint/RConn3 -- j27_Velocity/LConn1
  j28_Torque/RConn1 -- waist_roll_joint/LConn2
  waist_roll_joint/RConn3 -- j28_Velocity/LConn1
  j29_Torque/RConn1 -- waist_yaw_joint/LConn2
  waist_yaw_joint/RConn2 -- j29_Position/LConn1
  waist_yaw_joint/RConn3 -- j29_Velocity/LConn1
  d435_joint/RConn1 -- d435_link/LConn1
  head_joint/RConn1 -- head_link/LConn1
  left_hip_pitch_link/RConn1 -- left_hip_roll_joint/LConn1
  left_hip_roll_joint/RConn1 -- left_hip_roll_link/LConn1
  left_hip_roll_link/RConn1 -- left_hip_yaw_joint/LConn1
  left_hip_yaw_joint/RConn1 -- left_hip_yaw_link/LConn1
  left_hip_yaw_link/RConn1 -- left_knee_joint/LConn1
  left_knee_joint/RConn1 -- left_knee_link/LConn1
  left_ankle_pitch_joint/LConn1 -- left_knee_link/RConn1
  left_hand_palm_joint/RConn1 -- left_rubber_hand/LConn1
  left_shoulder_pitch_joint/RConn1 -- left_shoulder_pitch_link/LConn1
  left_shoulder_pitch_link/RConn1 -- left_shoulder_roll_joint/LConn1
  imu_in_pelvis/LConn1 -- imu_in_pelvis_joint/RConn1
  left_shoulder_roll_joint/RConn1 -- left_shoulder_roll_link/LConn1
  left_shoulder_roll_link/RConn1 -- left_shoulder_yaw_joint/LConn1
  left_shoulder_yaw_joint/RConn1 -- left_shoulder_yaw_link/LConn1
  left_elbow_joint/LConn1 -- left_shoulder_yaw_link/RConn1
  left_wrist_pitch_joint/RConn1 -- left_wrist_pitch_link/LConn1
  left_wrist_pitch_link/RConn1 -- left_wrist_yaw_joint/LConn1
  left_wrist_roll_joint/RConn1 -- left_wrist_roll_link/LConn1
  left_wrist_pitch_joint/LConn1 -- left_wrist_roll_link/RConn1
  left_wrist_yaw_joint/RConn1 -- left_wrist_yaw_link/LConn1
  left_hand_palm_joint/LConn1 -- left_wrist_yaw_link/RConn1
  imu_in_torso/LConn1 -- imu_in_torso_joint/RConn1
  logo_joint/RConn1 -- logo_link/LConn1
  mid360_joint/RConn1 -- mid360_link/LConn1
  pelvis_contour_joint/RConn1 -- pelvis_contour_link/LConn1
  right_ankle_pitch_joint/RConn1 -- right_ankle_pitch_link/LConn1
  right_ankle_pitch_link/RConn1 -- right_ankle_roll_joint/LConn1
  left_ankle_pitch_joint/RConn1 -- left_ankle_pitch_link/LConn1
  right_ankle_roll_joint/RConn1 -- right_ankle_roll_link/LConn1
  right_elbow_joint/RConn1 -- right_elbow_link/LConn1
  right_elbow_link/RConn1 -- right_wrist_roll_joint/LConn1
  right_hip_pitch_joint/RConn1 -- right_hip_pitch_link/LConn1
  right_hip_pitch_link/RConn1 -- right_hip_roll_joint/LConn1
  right_hip_roll_joint/RConn1 -- right_hip_roll_link/LConn1
  right_hip_roll_link/RConn1 -- right_hip_yaw_joint/LConn1
  right_hip_yaw_joint/RConn1 -- right_hip_yaw_link/LConn1
  right_hip_yaw_link/RConn1 -- right_knee_joint/LConn1
  right_knee_joint/RConn1 -- right_knee_link/LConn1
  left_ankle_pitch_link/RConn1 -- left_ankle_roll_joint/LConn1
  right_ankle_pitch_joint/LConn1 -- right_knee_link/RConn1
  right_hand_palm_joint/RConn1 -- right_rubber_hand/LConn1
  right_shoulder_pitch_joint/RConn1 -- right_shoulder_pitch_link/LConn1
  right_shoulder_pitch_link/RConn1 -- right_shoulder_roll_joint/LConn1
  right_shoulder_roll_joint/RConn1 -- right_shoulder_roll_link/LConn1
  right_shoulder_roll_link/RConn1 -- right_shoulder_yaw_joint/LConn1
  right_shoulder_yaw_joint/RConn1 -- right_shoulder_yaw_link/LConn1
  right_elbow_joint/LConn1 -- right_shoulder_yaw_link/RConn1
  right_wrist_pitch_joint/RConn1 -- right_wrist_pitch_link/LConn1
  right_wrist_pitch_link/RConn1 -- right_wrist_yaw_joint/LConn1
  left_ankle_roll_joint/RConn1 -- left_ankle_roll_link/LConn1
  right_wrist_roll_joint/RConn1 -- right_wrist_roll_link/LConn1
  right_wrist_pitch_joint/LConn1 -- right_wrist_roll_link/RConn1
  right_wrist_yaw_joint/RConn1 -- right_wrist_yaw_link/LConn1
  right_hand_palm_joint/LConn1 -- right_wrist_yaw_link/RConn1
  torso_link/LConn1 -- waist_pitch_joint/RConn1
  d435_joint/LConn1 -- torso_link/RConn8
  head_joint/LConn1 -- torso_link/RConn7
  imu_in_torso_joint/LConn1 -- torso_link/RConn6
  left_shoulder_pitch_joint/LConn1 -- torso_link/RConn5
  logo_joint/LConn1 -- torso_link/RConn4
  left_elbow_joint/RConn1 -- left_elbow_link/LConn1
  mid360_joint/LConn1 -- torso_link/RConn3
  right_shoulder_pitch_joint/LConn1 -- torso_link/RConn2
  torso_link/RConn1 -- waist_support_joint/LConn1
  waist_roll_joint/RConn1 -- waist_roll_link/LConn1
  waist_pitch_joint/LConn1 -- waist_roll_link/RConn1
  waist_support_joint/RConn1 -- waist_support_link/LConn1
  waist_yaw_joint/RConn1 -- waist_yaw_link/LConn1
  waist_roll_joint/LConn1 -- waist_yaw_link/RConn1
  left_elbow_link/RConn1 -- left_wrist_roll_joint/LConn1
  left_hip_pitch_joint/RConn1 -- left_hip_pitch_link/LConn1
  Ground/RConn1 -- LeftFootContact/LConn1 -- RightFootContact/LConn1
  World/RConn1 -- pelvis_Sensor/LConn1 -- FloatingBase/LConn1 -- Solver_Configuration/RConn1 -- MechanismConfiguration/RConn1 -- Ground/LConn1
  foot_r_contact_Sensor/RConn1 -- RightFootContact/RConn1 -- foot_r_contact/RConn1
  foot_l_contact/RConn1 -- foot_l_contact_Sensor/RConn1 -- LeftFootContact/RConn1
  right_wrist_roll_joint/RConn2 -- j25_Position/LConn1
  left_wrist_roll_joint/RConn3 -- j12_Velocity/LConn1
  right_ankle_roll_link/RConn1 -- foot_r_contact/LConn1
  left_ankle_roll_link/RConn1 -- foot_l_contact/LConn1
